simulink model "PV_SYSTEM_WITH_VARIOUS_MPPT"  (R2017a)
(part 4 of 6)

Inventec Energy IECS-6P68-190 | Inventec Energy IECS-6P69-190 | Inventec Energy IECS-6M68-195 | Inventec Energy IECS-6P68-195 | Inventec Energy IECS-6P69-195 | Inventec Energy IECS-6M69-200 | Inventec Energy IECS-6P68-200 | Inventec Energy IECS-6P69-200 | Inventec Energy IECS-6M69-205 | Inventec Energy IECS-6P68-205 | Inventec Energy IECS-6P69-205 | Inventec Energy IECS-6M69-210 | Inventec Energy IECS-6P69-210 | Inventec Energy IECS-6P6A-210 | Inventec Energy IECS-6M6A-215 | Inventec Energy IECS-6P69-215 | Inventec Energy IECS-6P6A-215 | Inventec Energy IECS-6M6A-220 | Inventec Energy IECS-6P69-220 | Inventec Energy IECS-6P6A-220 | Inventec Energy IECS-6M6A-225 | Inventec Energy IECS-6P69-225 | Inventec Energy IECS-6P6A-225 | Inventec Energy IECS-6M6A-230 | Inventec Energy IECS-6P69-230 | Inventec Energy IECS-6P6A-230 | Inventec Energy IECS-6M6A-235 | Inventec Energy IECS-6P6A-235 | Inventec Energy IECS-6M6A-240 | Inventec Energy IECS-6P6A-240 | Inventec Energy IECS-6M6A-245 | Inventec Energy IECS-6P6A-245 | Inventec Energy IECS-6M6A-250 | Inventec Energy IECS-6P6A-250 | Inventec Energy IECS-6M6A-255 | Inventec Energy IECS-6P6A-255 | Inventec Energy IECS-6M6A-260 | Inventec Energy IECS-6M6A-265 | Inventec Energy IECS-6M6A-270 | Inventec Energy IECS-6M6A-275 | Inventec Energy IECS-6P6C-275 | Inventec Energy IECS-6P6C-280 | Inventec Energy IECS-6M6C-285 | Inventec Energy IECS-6P6C-285 | Inventec Energy IECS-6M6C-290 | Inventec Energy IECS-6P6C-290 | Inventec Energy IECS-6M6C-295 | Inventec Energy IECS-6P6C-295 | Inventec Energy IECS-6M6C-300 | Inventec Energy IECS-6P6C-300 | Inventec Energy IECS-6M6C-305 | Inventec Energy IECS-6M6C-310 | Inventec Energy IECS-6M6C-315 | Inventec Energy IECS-6M6C-320 | Inventec Energy IECS-6M6C-325 | Inventec Energy IECS-6M6C-330 | Isofoton IS-210-32 | Isofoton IS-215-32 | Isofoton IS-220-32 | Isofoton ISF-235 | Isofoton ISF-240 | Isofoton ISF-245 | Isofoton ISF-245 Black | Isofoton ISF-245 Clear | Isofoton ISFT-245 | Isofoton ISF-250 | Isofoton ISF-250 Black | Isofoton ISF-250 Clear | Isofoton ISFT-250 | Isofoton ISF-255 | Isofoton ISF-255 Black | Isofoton ISF-255 Clear | Isofoton ISFT-255 | iTek iT-220 | iTek iT-225 | iTek iT-230 | iTek iT-235 | iTek iT-240 | Jetion Solar (China) JT175SAb | Jetion Solar (China) JT175SAb(Black) | Jetion Solar (China) JT180SAb | Jetion Solar (China) JT180SAb(Black) | Jetion Solar (China) JT185SAb | Jetion Solar (China) JT185SAb(Black) | Jetion Solar (China) JT190SAb | Jetion Solar (China) JT195SAb | Jetion Solar (China) JT220PCe | Jetion Solar (China) JT220PCe(Black) | Jetion Solar (China) JT225PCe | Jetion Solar (China) JT225PCe(Black) | Jetion Solar (China) JT230PCe | Jetion Solar (China) JT230PCe(Black) | Jetion Solar (China) JT230SCc | Jetion Solar (China) JT230SCc(Black) | Jetion Solar (China) JT235PCe | Jetion Solar (China) JT235PCe(Black) | Jetion Solar (China) JT235SCc | Jetion Solar (China) JT235SCc(Black) | Jetion Solar (China) JT240PCe | Jetion Solar (China) JT240PCe(Black) | Jetion Solar (China) JT240SCc | Jetion Solar (China) JT240SCc(Black) | Jetion Solar (China) JT245SCc | Jetion Solar (China) JT245SCc(Black) | Jetion Solar (China) JT250SCc | Jetion Solar (China) JT270PAe | Jetion Solar (China) JT270PAe(Black) | Jetion Solar (China) JT270SAc | Jetion Solar (China) JT270SAc(Black) | Jetion Solar (China) JT275PAe | Jetion Solar (China) JT275PAe(Black) | Jetion Solar (China) JT275SAc | Jetion Solar (China) JT275SAc(Black) | Jetion Solar (China) JT280PAe | Jetion Solar (China) JT280PAe(Black) | Jetion Solar (China) JT280SAc | Jetion Solar (China) JT280SAc(Black) | Jetion Solar (China) JT285PAe | Jetion Solar (China) JT285PAe(Black) | Jetion Solar (China) JT285SAc | Jetion Solar (China) JT285SAc(Black) | Jetion Solar (China) JT290PAe | Jetion Solar (China) JT290PAe(Black) | Jetion Solar (China) JT290SAc | Jetion Solar (China) JT290SAc(Black) | Jiangsu Aide Solar Energy Technology AD160M5-Aa | Jiangsu Aide Solar Energy Technology AD165M5-Aa | Jiangsu Aide Solar Energy Technology AD170M5-Aa | Jiangsu Aide Solar Energy Technology AD175M5-Aa | Jiangsu Aide Solar Energy Technology AD180M5-Aa | Jiangsu Aide Solar Energy Technology AD185M5-Aa | Jiangsu Aide Solar Energy Technology AD190M5-Aa | Jiangsu Aide Solar Energy Technology AD190P6-Ac | Jiangsu Aide Solar Energy Technology AD195M5-Aa | Jiangsu Aide Solar Energy Technology AD195P6-Ac | Jiangsu Aide Solar Energy Technology AD200M5-Aa | Jiangsu Aide Solar Energy Technology AD200P6-Ac | Jiangsu Aide Solar Energy Technology AD205P6-Ac | Jiangsu Aide Solar Energy Technology AD210P6-Ac | Jiangsu Aide Solar Energy Technology AD210P6-Bc | Jiangsu Aide Solar Energy Technology AD215P6-Ab | Jiangsu Aide Solar Energy Technology AD220P6-Ab | Jiangsu Aide Solar Energy Technology AD220P6-Bb | Jiangsu Aide Solar Energy Technology AD225P6-Ab | Jiangsu Aide Solar Energy Technology AD230M6-Ab | Jiangsu Aide Solar Energy Technology AD230P6-Ab | Jiangsu Aide Solar Energy Technology AD230P6-Bb | Jiangsu Aide Solar Energy Technology AD235M6-Ab | Jiangsu Aide Solar Energy Technology AD235P6-Ab | Jiangsu Aide Solar Energy Technology AD235P6-Bb | Jiangsu Aide Solar Energy Technology AD240M6-Ab | Jiangsu Aide Solar Energy Technology AD240P6-Ab | Jiangsu Aide Solar Energy Technology AD240P6-Bb | Jiangsu Aide Solar Energy Technology AD245M6-Ab | Jiangsu Aide Solar Energy Technology AD245P6-Ab | Jiangsu Aide Solar Energy Technology AD250M6-Ab | Jiangsu Aide Solar Energy Technology AD250P6-Ab | Jiangsu Aide Solar Energy Technology AD255M6-Ab | Jiangsu Aide Solar Energy Technology AD255P6-Ab | Jiangsu Aide Solar Energy Technology AD260M6-Ab | Jiangsu Aide Solar Energy Technology AD260P6-Ab | Jiangsu Aide Solar Energy Technology AD265M6-Ab | Jiangsu Aide Solar Energy Technology AD275M6-Aa | Jiangsu Aide Solar Energy Technology AD275P6-Aa | Jiangsu Aide Solar Energy Technology AD280M6-Aa | Jiangsu Aide Solar Energy Technology AD280P6-Aa | Jiangsu Aide Solar Energy Technology AD285M6-Aa | Jiangsu Aide Solar Energy Technology AD285P6-Aa | Jiangsu Aide Solar Energy Technology AD290M6-Aa | Jiangsu Aide Solar Energy Technology AD290P6-Aa | Jiangsu Aide Solar Energy Technology AD295M6-Aa | Jiangsu Aide Solar Energy Technology AD295P6-Aa | Jiangsu Aide Solar Energy Technology AD300M6-Aa | Jiangsu Aide Solar Energy Technology AD300P6-Aa | Jiangsu Aide Solar Energy Technology AD305M6-Aa | Jiangsu Aide Solar Energy Technology AD305P6-Aa | Jiangsu Aide Solar Energy Technology AD310M6-Aa | Jiangsu Aide Solar Energy Technology AD310P6-Aa | Jiangsu Aide Solar Energy Technology AD315M6-Aa | Jiangsu Best Solar High-Tech BEST-170D-24 | Jiangsu Best Solar High-Tech BEST-175D-24 | Jiangsu Best Solar High-Tech BEST-180D-24 | Jiangsu Best Solar High-Tech BEST-190P-18 | Jiangsu Best Solar High-Tech BEST-200P-18 | Jiangsu Best Solar High-Tech BEST-210P-18 | Jiangsu Best Solar High-Tech BEST-210P-20 | Jiangsu Best Solar High-Tech BEST-220D-20 | Jiangsu Best Solar High-Tech BEST-220P-20 | Jiangsu Best Solar High-Tech BEST-230D-20 | Jiangsu Best Solar High-Tech BEST-230P-20 | Jiangsu Best Solar High-Tech BEST-240D-20 | Jiangsu Best Solar High-Tech BEST-260P-24 | Jiangsu Best Solar High-Tech BEST-270P-24 | Jiangsu Best Solar High-Tech BEST-280P-24 | Jiangsu Green Power PV GPM175-A-72 | Jiangsu Green Power PV GPM175-B-48 | Jiangsu Green Power PV GPM175P-B-48 | Jiangsu Green Power PV GPM180-A-72 | Jiangsu Green Power PV GPM180-B-48 | Jiangsu Green Power PV GPM180P-B-48 | Jiangsu Green Power PV GPM185-A-72 | Jiangsu Green Power PV GPM185-B-48 | Jiangsu Green Power PV GPM185P-B-48 | Jiangsu Green Power PV GPM190-B-54 | Jiangsu Green Power PV GPM190P-B-54 | Jiangsu Green Power PV GPM195-B-54 | Jiangsu Green Power PV GPM195P-B-54 | Jiangsu Green Power PV GPM200-B-54 | Jiangsu Green Power PV GPM200P-B-54 | Jiangsu Green Power PV GPM205-B-54 | Jiangsu Green Power PV GPM205P-B-54 | Jiangsu Green Power PV GPM210-B-54 | Jiangsu Green Power PV GPM210P-B-54 | Jiangsu Green Power PV GPM210P-B-60 | Jiangsu Green Power PV GPM215P-B-60 | Jiangsu Green Power PV GPM220-B-60 | Jiangsu Green Power PV GPM220P-B-60 | Jiangsu Green Power PV GPM225-B-60 | Jiangsu Green Power PV GPM225P-B-60 | Jiangsu Green Power PV GPM230-B-60 | Jiangsu Green Power PV GPM230P-B-60 | Jiangsu Green Power PV GPM235-B-60 | Jiangsu Green Power PV GPM240-B-60 | Jiangsu JiaSheng Photovoltaic Technology JS140M36-12V | Jiangsu JiaSheng Photovoltaic Technology JS140P36-12V | Jiangsu JiaSheng Photovoltaic Technology JS145M36-12V | Jiangsu JiaSheng Photovoltaic Technology JS145P36-12V | Jiangsu JiaSheng Photovoltaic Technology JS180D72-24V | Jiangsu JiaSheng Photovoltaic Technology JS185D72-24V | Jiangsu JiaSheng Photovoltaic Technology JS190D72-24V | Jiangsu JiaSheng Photovoltaic Technology JS195D72-24V | Jiangsu JiaSheng Photovoltaic Technology JS220P60-24V | Jiangsu JiaSheng Photovoltaic Technology JS225P60-24V | Jiangsu JiaSheng Photovoltaic Technology JS230M60-24V | Jiangsu JiaSheng Photovoltaic Technology JS230P60-24V | Jiangsu JiaSheng Photovoltaic Technology JS235M60-24V | Jiangsu JiaSheng Photovoltaic Technology JS235P60-24V | Jiangsu JiaSheng Photovoltaic Technology JS240M60-24V | Jiangsu JiaSheng Photovoltaic Technology JS240P60-24V | Jiangsu JiaSheng Photovoltaic Technology JS245M60-24V | Jiangsu JiaSheng Photovoltaic Technology JS250M60-24V | Jiangsu JiaSheng Photovoltaic Technology JS255M60-24V | Jiangsu JiaSheng Photovoltaic Technology JS255P72-24V | Jiangsu JiaSheng Photovoltaic Technology JS260M60-24V | Jiangsu JiaSheng Photovoltaic Technology JS260M72-24V | Jiangsu JiaSheng Photovoltaic Technology JS260P72-24V | Jiangsu JiaSheng Photovoltaic Technology JS265M72-24V | Jiangsu JiaSheng Photovoltaic Technology JS265P72-24V | Jiangsu JiaSheng Photovoltaic Technology JS270M72-24V | Jiangsu JiaSheng Photovoltaic Technology JS270P72-24V | Jiangsu JiaSheng Photovoltaic Technology JS275M72-24V | Jiangsu JiaSheng Photovoltaic Technology JS275P72-24V | Jiangsu JiaSheng Photovoltaic Technology JS280M72-24V | Jiangsu JiaSheng Photovoltaic Technology JS280P72-24V | Jiangsu JiaSheng Photovoltaic Technology JS290M72-24V | Jiangsu JiaSheng Photovoltaic Technology JS290P72-24V | Jiangsu JiaSheng Photovoltaic Technology JS300M72-24V | Jiangsu JiaSheng Photovoltaic Technology JS300P72-24V | Jiangsu Prefersolar Photovoltaic PS-175M | Jiangsu Prefersolar Photovoltaic PS-180M | Jiangsu Prefersolar Photovoltaic PS-185M | Jiangsu Prefersolar Photovoltaic PS-230M | Jiangsu Prefersolar Photovoltaic PS-235M | Jiangsu Prefersolar Photovoltaic PS-240M | Jiangsu Prefersolar Photovoltaic PS-245M | Jiangsu Prefersolar Photovoltaic PS-250M | Jiangsu Runda PV RS185M-72 | Jiangsu Runda PV RS190M-72 | Jiangsu Runda PV RS215P-60 | Jiangsu Runda PV RS220P-60 | Jiangsu Runda PV RS225P-60 | Jiangsu Runda PV RS230M-96 | Jiangsu Runda PV RS230P-60 | Jiangsu Runda PV RS235M-96 | Jiangsu Runda PV RS235P-60 | Jiangsu Runda PV RS240M-96 | Jiangsu Runda PV RS245M-96 | Jiangsu Runda PV RS250M-96 | Jiangsu Sainty Machinery GES-M165 | Jiangsu Sainty Machinery GES-5M170 | Jiangsu Sainty Machinery GES-M170 | Jiangsu Sainty Machinery GES-5M175 | Jiangsu Sainty Machinery GES-M175 | Jiangsu Sainty Machinery GES-5M180 | Jiangsu Sainty Machinery GES-M180 | Jiangsu Sainty Machinery GES-5M185 | Jiangsu Sainty Machinery GES-5M190 | Jiangsu Sainty Machinery GES-6M190 | Jiangsu Sainty Machinery GES-5M195 | Jiangsu Sainty Machinery GES-6M195 | Jiangsu Sainty Machinery GES-6M200 | Jiangsu Sainty Machinery GES-P200 | Jiangsu Sainty Machinery GES-6M205 | Jiangsu Sainty Machinery GES-6M210 | Jiangsu Sainty Machinery GES-P210 | Jiangsu Sainty Machinery GES-6M220 | Jiangsu Sainty Machinery GES-P220 | Jiangsu Sainty Machinery GES-6M225 | Jiangsu Sainty Machinery GES-6P225 | Jiangsu Sainty Machinery GES-5M230 | Jiangsu Sainty Machinery GES-6M230 | Jiangsu Sainty Machinery GES-6P230 | Jiangsu Sainty Machinery GES-P230 | Jiangsu Sainty Machinery GES-5M235 | Jiangsu Sainty Machinery GES-6M235 | Jiangsu Sainty Machinery GES-6P235 | Jiangsu Sainty Machinery GES-5M240 | Jiangsu Sainty Machinery GES-6M240 | Jiangsu Sainty Machinery GES-6P240 | Jiangsu Sainty Machinery GES-P240 | Jiangsu Sainty Machinery GES-5M245 | Jiangsu Sainty Machinery GES-6M245 | Jiangsu Sainty Machinery GES-6P245 | Jiangsu Sainty Machinery GES-5M250 | Jiangsu Sainty Machinery GES-6M250 | Jiangsu Sainty Machinery GES-P250 | Jiangsu Sainty Machinery GES-5M255 | Jiangsu Sainty Machinery GES-6M255 | Jiangsu Sainty Machinery GES-6P255 | Jiangsu Sainty Machinery GES-6M260 | Jiangsu Sainty Machinery GES-6P260 | Jiangsu Sainty Machinery GES-P260 | Jiangsu Sainty Machinery GES-6M265 | Jiangsu Sainty Machinery GES-6P265 | Jiangsu Sainty Machinery GES-6M270 | Jiangsu Sainty Machinery GES-6P270 | Jiangsu Sainty Machinery GES-P270 | Jiangsu Sainty Machinery GES-6M275 | Jiangsu Sainty Machinery GES-6P275 | Jiangsu Sainty Machinery GES-6M280 | Jiangsu Sainty Machinery GES-6P280 | Jiangsu Sainty Machinery GES-P280 | Jiangsu Sainty Machinery GES-6M285 | Jiangsu Sainty Machinery GES-6P285 | Jiangsu Sainty Machinery GES-6M290 | Jiangsu Sainty Machinery GES-6P290 | Jiangsu Sainty Machinery GES-6M295 | Jiangsu Sainty Machinery GES-6P295 | Jiangsu Sainty Machinery GES-6M300 | Jiangsu Sainty Machinery GES-6P300 | Jiangsu Sainty Machinery GES-6M305 | Jiangsu Sainty Machinery GES-6M310 | Jiangsu Sainty Machinery GES-6M315 | Jiangsu Shunda PV-Tech SDM-170-(165)-72M | Jiangsu Shunda PV-Tech SDM-170-(170)-72M | Jiangsu Shunda PV-Tech SDM-170-(175)-72M | Jiangsu Shunda PV-Tech SDM-170-(180)-72M | Jiangsu Shunda PV-Tech SDM-170-(185)-72M | Jiangsu SunLink PV Technology SL180-24M170 | Jiangsu SunLink PV Technology SL180-24M175 | Jiangsu SunLink PV Technology SL180-24M180 | Jiangsu SunLink PV Technology SL180-24M185 | Jiangsu SunLink PV Technology SL180-24M190 | Jiangsu SunLink PV Technology SL180-24M195 | Jiangsu SunLink PV Technology SL220-20M200 | Jiangsu SunLink PV Technology SL220-20P200 | Jiangsu SunLink PV Technology SL220-20M205 | Jiangsu SunLink PV Technology SL220-20P205 | Jiangsu SunLink PV Technology SL220-20M210 | Jiangsu SunLink PV Technology SL220-20P210 | Jiangsu SunLink PV Technology SL220-20M215 | Jiangsu SunLink PV Technology SL220-20P215 | Jiangsu SunLink PV Technology SL220-20M220 | Jiangsu SunLink PV Technology SL220-20P220 | Jiangsu SunLink PV Technology SL240-32M220 | Jiangsu SunLink PV Technology SL220-20M225 | Jiangsu SunLink PV Technology SL220-20P225 | Jiangsu SunLink PV Technology SL240-32M225 | Jiangsu SunLink PV Technology SL220-20M230 | Jiangsu SunLink PV Technology SL220-20P230 | Jiangsu SunLink PV Technology SL240-32M230 | Jiangsu SunLink PV Technology SL220-20M235 | Jiangsu SunLink PV Technology SL220-20P235 | Jiangsu SunLink PV Technology SL240-32M235 | Jiangsu SunLink PV Technology SL220-20M240 | Jiangsu SunLink PV Technology SL220-20P240 | Jiangsu SunLink PV Technology SL240-32M240 | Jiangsu SunLink PV Technology SL220-20M245 | Jiangsu SunLink PV Technology SL240-32M245 | Jiangsu SunLink PV Technology SL220-20M250 | Jiangsu SunLink PV Technology SL240-32M250 | Jiangsu SunLink PV Technology SL220-20M255 | Jiangsu SunLink PV Technology SL240-32M255 | Jiangsu SunLink PV Technology SL220-20M260 | Jiangsu SunLink PV Technology SL280-24M260 | Jiangsu SunLink PV Technology SL280-24P260 | Jiangsu SunLink PV Technology SL280-24M265 | Jiangsu SunLink PV Technology SL280-24P265 | Jiangsu SunLink PV Technology SL280-24M270 | Jiangsu SunLink PV Technology SL280-24P270 | Jiangsu SunLink PV Technology SL280-24M275 | Jiangsu SunLink PV Technology SL280-24P275 | Jiangsu SunLink PV Technology SL280-24M280 | Jiangsu SunLink PV Technology SL280-24P280 | Jiangsu SunLink PV Technology SL280-24M285 | Jiangsu SunLink PV Technology SL280-24P285 | Jiangsu SunLink PV Technology SL280-24M290 | Jiangsu SunLink PV Technology SL280-24P290 | Jiangsu SunLink PV Technology SL280-24M295 | Jiangsu SunLink PV Technology SL280-24P295 | Jiangsu Wanfeng PV WF175M-01E | Jiangsu Wanfeng PV WF180M-01E | Jiangsu Wanfeng PV WF185M-01E | Jiangsu Wanfeng PV WF200P-02B | Jiangsu Wanfeng PV WF205P-02B | Jiangsu Wanfeng PV WF210P-02B | Jiangsu Wanfeng PV WF215P-02B | Jiangsu Wanfeng PV WF220P-02B | Jiangsu Wanfeng PV WF225P-02B | Jiangsu Wanfeng PV WF230P-02B | Jiangsu Wanfeng PV WF240P-02A | Jiangsu Wanfeng PV WF245P-02A | Jiangsu Wanfeng PV WF250P-02A | Jiangsu Wanfeng PV WF255P-02A | Jiangsu Wanfeng PV WF260P-02A | Jiangsu Wanfeng PV WF265P-02A | Jiangsu Wanfeng PV WF270P-02A | Jiangsu Wanfeng PV WF275P-02A | Jiangsu Wanfeng PV WF280P-02A | Jiangxi Best Solar High-Tech BEST-170D-24 | Jiangxi Best Solar High-Tech BEST-175D-24 | Jiangxi Best Solar High-Tech BEST-180D-24 | Jiangxi Best Solar High-Tech BEST-190P-18 | Jiangxi Best Solar High-Tech BEST-200P-18 | Jiangxi Best Solar High-Tech BEST-210P-18 | Jiangxi Best Solar High-Tech BEST-210P-20 | Jiangxi Best Solar High-Tech BEST-220D-20 | Jiangxi Best Solar High-Tech BEST-220P-20 | Jiangxi Best Solar High-Tech BEST-230D-20 | Jiangxi Best Solar High-Tech BEST-230P-20 | Jiangxi Best Solar High-Tech BEST-240D-20 | Jiangxi Best Solar High-Tech BEST-260P-24 | Jiangxi Best Solar High-Tech BEST-270P-24 | Jiangxi Best Solar High-Tech BEST-280P-24 | Jiangyin Hareon Power HR-115W-17V | Jiangyin Hareon Power HR-120W-17V | Jiangyin Hareon Power HR-125W-17V | Jiangyin Hareon Power HR-160W-24V | Jiangyin Hareon Power HR-165W-24V | Jiangyin Hareon Power HR-170W-24V | Jiangyin Hareon Power HR-175W-24V | Jiangyin Hareon Power HR-180W-24V | Jiangyin Hareon Power HR-185W-24V | Jiangyin Hareon Power HR-190W-24V | Jiangyin Hareon Power HR-195W-24V | Jiangyin Hareon Power HR-200W-18V | Jiangyin Hareon Power HR-200W-24V | Jiangyin Hareon Power HR-205W-18V | Jiangyin Hareon Power HR-210W-18V | Jiangyin Hareon Power HR-215W-18V | Jiangyin Hareon Power HR220D6P-3 | Jiangyin Hareon Power HR-220W-18V | Jiangyin Hareon Power HR225D6P-3 | Jiangyin Hareon Power HR-225P-18-Bb | Jiangyin Hareon Power HR-225P-18-Bbp | Jiangyin Hareon Power HR-225W-18V | Jiangyin Hareon Power HR230D6P-3 | Jiangyin Hareon Power HR-230P-18-Bb | Jiangyin Hareon Power HR-230P-18-Bbp | Jiangyin Hareon Power HR-230W-18V | Jiangyin Hareon Power HR235D6P-3 | Jiangyin Hareon Power HR-235P-18-Bb | Jiangyin Hareon Power HR-235P-18-Bbp | Jiangyin Hareon Power HR-235W-18V | Jiangyin Hareon Power HR-240P-18-Bb | Jiangyin Hareon Power HR-240P-18-Bbp | Jiangyin Hareon Power HR-240W-18V | Jiangyin Hareon Power HR-245P-18-Bb | Jiangyin Hareon Power HR-245P-18-Bbp | Jiangyin Hareon Power HR-250-18-Cb | Jiangyin Hareon Power HR-250P-18-Bb | Jiangyin Hareon Power HR-250P-18-Bbp | Jiangyin Hareon Power HR-255-18-Cb | Jiangyin Hareon Power HR-255P-18-Bb | Jiangyin Hareon Power HR-255P-18-Bbp | Jiangyin Hareon Power HR-260-18-Cb | Jiangyin Hareon Power HR-260P-18-Bb | Jiangyin Hareon Power HR-260P-18-Bbp | Jiangyin Hareon Power HR-265-18-Cb | Jiangyin Hareon Power HR-265P-18-Bb | Jiangyin Hareon Power HR-265P-18-Bbp | Jiangyin Hareon Power HR-270-18-Cb | Jiangyin Hareon Power HR-270P-24-Ba | Jiangyin Hareon Power HR-270P-24-Bap | Jiangyin Hareon Power HR-275P-24-Ba | Jiangyin Hareon Power HR-275P-24-Bap | Jiangyin Hareon Power HR-280P-24-Ba | Jiangyin Hareon Power HR-280P-24-Bap | Jiangyin Hareon Power HR-285P-24-Ba | Jiangyin Hareon Power HR-285P-24-Bap | Jiangyin Hareon Power HR-290P-24-Ba | Jiangyin Hareon Power HR-290P-24-Bap | Jiangyin Hareon Power HR-295-24-Ca | Jiangyin Hareon Power HR-295P-24-Ba | Jiangyin Hareon Power HR-295P-24-Bap | Jiangyin Hareon Power HR-300-24-Ca | Jiangyin Hareon Power HR-300P-24-Ba | Jiangyin Hareon Power HR-300P-24-Bap | Jiangyin Hareon Power HR-305-24-Ca | Jiangyin Hareon Power HR-305P-24-Ba | Jiangyin Hareon Power HR-305P-24-Bap | Jiangyin Hareon Power HR-310-24-Ca | Jiangyin Hareon Power HR-310P-24-Ba | Jiangyin Hareon Power HR-310P-24-Bap | Jiangyin Hareon Power HR-315-24-Ca | Jiangyin Hareon Power HR-315P-24-Ba | Jiangyin Hareon Power HR-315P-24-Bap | Jiangyin Hareon Power HR-320P-24-Ba | Jiangyin Hareon Power HR-320P-24-Bap | Jiangyin Jetion Science and Technology JT210PCe | Jiangyin Jetion Science and Technology JT215PCe | Jiawei Solarchina (Shenzhen) JW-G2300-MD6660P-1 | Jiawei Solarchina (Shenzhen) JW-G2300-QC6660P-1 | Jingao Solar JAM5(L)-175 | Jingao Solar JAM5(L)-180 | Jingao Solar JAM5(L)-185 | Jingao Solar JAM6-200 | Jingao Solar JAP6-200 | Jingao Solar JAM6-205 | Jingao Solar JAP6-205 | Jingao Solar JAM6-210 | Jingao Solar JAP6-210 | Jingao Solar JAM6-215 | Jingao Solar JAP6-215 | Jingao Solar JAM6-220 | Jingao Solar JAP6-220 | Jingao Solar JAM6-225 | Jingao Solar JAP6-225 | Jingao Solar JAM6-230 | Jingao Solar JAP6-230 | Jingao Solar JAM6-235 | Jingao Solar JAP6-235 | Jingao Solar JAM6-240 | Jingao Solar JAP6-240 | Jinko Solar JKM170M-72B | Jinko Solar JKM175M-72 | Jinko Solar JKM175M-72B | Jinko Solar JKM180M-72 | Jinko Solar JKM180M-72B | Jinko Solar JKM185M-72 | Jinko Solar JKM185M-72B | Jinko Solar JKM190M-72 | Jinko Solar JKM190M-72B | Jinko Solar JKM195M-72 | Jinko Solar JKM195M-72B | Jinko Solar JKM200M-60B | Jinko Solar JKM200M-72 | Jinko Solar JKM200M-72B | Jinko Solar JKM200P-60B | Jinko Solar JKM205M-60B | Jinko Solar JKM205M-72 | Jinko Solar JKM205M-72B | Jinko Solar JKM205P-60B | Jinko Solar JKM210M-60B | Jinko Solar JKM210P-60B | Jinko Solar JKM215M-60B | Jinko Solar JKM215P-60B | Jinko Solar JKM220M-60 | Jinko Solar JKM220M-60B | Jinko Solar JKM220P-60 | Jinko Solar JKM220P-60B | Jinko Solar JKM225M-60 | Jinko Solar JKM225M-60B | Jinko Solar JKM225P-60 | Jinko Solar JKM225P-60B | Jinko Solar JKM230M-60 | Jinko Solar JKM230M-60B | Jinko Solar JKM230P-60 | Jinko Solar JKM230P-60B | Jinko Solar JKM235M-60 | Jinko Solar JKM235M-60B | Jinko Solar JKM235P-60 | Jinko Solar JKM235P-60B | Jinko Solar JKM240M-60 | Jinko Solar JKM240M-60B | Jinko Solar JKM240P-60 | Jinko Solar JKM240P-60B | Jinko Solar JKM245M-60 | Jinko Solar JKM245M-60B | Jinko Solar JKM245P-60 | Jinko Solar JKM245P-60B | Jinko Solar JKM250M-60 | Jinko Solar JKM250M-72B | Jinko Solar JKM250P-60 | Jinko Solar JKM250P-72 | Jinko Solar JKM250P-72B | Jinko Solar JKM255M-60 | Jinko Solar JKM255M-72B | Jinko Solar JKM255M-96 | Jinko Solar JKM255P-60 | Jinko Solar JKM255P-72 | Jinko Solar JKM255P-72B | Jinko Solar JKM260M-72B | Jinko Solar JKM260M-96 | Jinko Solar JKM260P-72 | Jinko Solar JKM260P-72B | Jinko Solar JKM265M-72B | Jinko Solar JKM265M-96 | Jinko Solar JKM265P-72 | Jinko Solar JKM265P-72B | Jinko Solar JKM270M-72 | Jinko Solar JKM270M-72B | Jinko Solar JKM270M-96 | Jinko Solar JKM270P-72 | Jinko Solar JKM270P-72B | Jinko Solar JKM275M-72 | Jinko Solar JKM275M-72B | Jinko Solar JKM275M-96 | Jinko Solar JKM275P-72 | Jinko Solar JKM275P-72B | Jinko Solar JKM280M-72 | Jinko Solar JKM280M-72B | Jinko Solar JKM280M-96 | Jinko Solar JKM280P-72 | Jinko Solar JKM280P-72B | Jinko Solar JKM285M-72 | Jinko Solar JKM285M-72B | Jinko Solar JKM285P-72 | Jinko Solar JKM285P-72B | Jinko Solar JKM290M-72 | Jinko Solar JKM290M-72B | Jinko Solar JKM290P-72 | Jinko Solar JKM290P-72B | Jinko Solar JKM295M-72 | Jinko Solar JKM295M-72B | Jinko Solar JKM295P-72 | Jinko Solar JKM295P-72B | Jinko Solar JKM300M-72 | Jinko Solar JKM305M-72 | Jinko Solar JKM305P-72 | Jinko Solar JKM310M-72 | Jinzhou Jinmao Photovoltaic Technology JMPV-5M-36-85 | Jinzhou Jinmao Photovoltaic Technology JMPV-5M-36-90 | Jinzhou Jinmao Photovoltaic Technology JMPV-5M-36-95 | Jinzhou Jinmao Photovoltaic Technology JMPV-5M-72-165 | Jinzhou Jinmao Photovoltaic Technology JMPV-5M-72-170 | Jinzhou Jinmao Photovoltaic Technology JMPV-5M-72-175 | Jinzhou Jinmao Photovoltaic Technology JMPV-5M-72-180 | Jinzhou Jinmao Photovoltaic Technology JMPV-5M-72-185 | Jinzhou Jinmao Photovoltaic Technology JMPV-5M-72-190 | Juli New Energy JLS155M | Juli New Energy JLS160M | Juli New Energy JLS165M | Juli New Energy JLS170M | Juli New Energy JLS175M | Juli New Energy JLS180M | Juli New Energy JLS200M | Juli New Energy JLS205M | Juli New Energy JLS210M | Juli New Energy JLS215P | Juli New Energy JLS220P | Juli New Energy JLS225P | Juli New Energy JLS230P | Jumao Photonic (Xiamen) JMP-85W-S5-G | Jumao Photonic (Xiamen) JMP-160W-S5-G | Jumao Photonic (Xiamen) JMP-170W-S5-G | Jumao Photonic (Xiamen) JMP-210W-M6-G | Jumao Photonic (Xiamen) JMP-215W-M6-G | Jumao Photonic (Xiamen) JMP-220W-M6-G | Jumao Photonic (Xiamen) JMP-225W-M6-G | Jumao Photonic (Xiamen) JMP-230W-M6-G | Kaneka G-SA060 | Kaneka GSA221 | Kaneka U-SA105 | Kaneka U-SA110 | KD Solar KD-20012A2 | KD Solar KD-20013A2 | KD Solar KD-20512A2 | KD Solar KD-20513A2 | KD Solar KD-21012A2 | KD Solar KD-21013A2 | KD Solar KD-21512A2 | KD Solar KD-21513A2 | KD Solar KD-22012A2 | KD Solar KD-22013A2 | KD Solar KD-22512A2 | KD Solar KD-22513A2 | KD Solar KD-23012A2 | KD Solar KD-23013A2 | KD Solar KD-23512A2 | KD Solar KD-24012A2 | Kenmec Mechanical Engineering TKSE-13001 | Kenmec Mechanical Engineering TKSE-13501 | Kenmec Mechanical Engineering TKSE-14001 | Kenmec Mechanical Engineering TKSE-14501 | Kenmec Mechanical Engineering TKSD-15001 | Kenmec Mechanical Engineering TKSD-15501 | Kenmec Mechanical Engineering TKSD-16001 | Kenmec Mechanical Engineering TKSD-16501 | Kenmec Mechanical Engineering TKSC-17001 | Kenmec Mechanical Engineering TKSD-17001 | Kenmec Mechanical Engineering TKSC-17501 | Kenmec Mechanical Engineering TKSC-18001 | Kenmec Mechanical Engineering TKSC-18501 | Kenmec Mechanical Engineering TKSC-19001 | Kenmec Mechanical Engineering TKSC-19501 | Kenmec Mechanical Engineering TKSB-20001 | Kenmec Mechanical Engineering TKSB-20501 | Kenmec Mechanical Engineering TKSB-21001 | Kenmec Mechanical Engineering TKSB-21501 | Kenmec Mechanical Engineering TKSA-22001 | Kenmec Mechanical Engineering TKSB-22001 | Kenmec Mechanical Engineering TKSA-22501 | Kenmec Mechanical Engineering TKSA-23001 | Kenmec Mechanical Engineering TKSA-23501 | Kenmec Mechanical Engineering TKSA-24001 | Kenmec Mechanical Engineering TKSA-24501 | Kenmec Mechanical Engineering TKSA-25001 | Kenmec Mechanical Engineering TKSG-25001 | Kenmec Mechanical Engineering TKSA-25501 | Kenmec Mechanical Engineering TKSG-25501 | Kenmec Mechanical Engineering TKSA-26001 | Kenmec Mechanical Engineering TKSG-26001 | Kenmec Mechanical Engineering TKSG-26501 | Kenmec Mechanical Engineering TKSG-27001 | Kenmec Mechanical Engineering TKSG-27501 | Kenmec Mechanical Engineering TKSG-28001 | Kenmec Mechanical Engineering TKSG-28501 | Kenmec Mechanical Engineering TKSG-29001 | Kenmec Mechanical Engineering TKSG-29501 | Kenmec Mechanical Engineering TKSG-30001 | Kenmec Mechanical Engineering TKSG-30501 | Kenmec Mechanical Engineering TKSG-31001 | Kenmec Mechanical Engineering TKSG-31501 | Kenmos Photovoltaic aTT-50W-02 | Kinve Solar Power KV170-72M | Kinve Solar Power KV175-72M | Kinve Solar Power KV180-72M | KISCO S91E | KISCO S92E | KISCO S93E | KISCO S94E | KISCO S95E | KISCO S96E | KISCO S97E | KISCO S98E | KISCO S99E | KISCO S100E | KISCO S101E | KISCO GETWATT 224P-A1U | KISCO GETWATT 225P-A1U | KISCO GETWATT 226P-A1U | KISCO GETWATT 227P-A1U | KISCO GETWATT 228P-A1U | KISCO GETWATT 229P-A1U | KISCO GETWATT 230P-A1U | KISCO GETWATT 231P-A1U | KISCO GETWATT 232P-A1U | KISCO GETWATT 233P-A1U | KISCO GETWATT 234P-A1U | KISCO GETWATT 235P-A1U | KISCO GETWATT 236P-A1U | KISCO GETWATT 237P-A1U | KISCO GETWATT 238M-A1U | KISCO GETWATT 238P-A1U | KISCO GETWATT 239M-A1U | KISCO GETWATT 239P-A1U | KISCO GETWATT 240M-A1U | KISCO GETWATT 240M-C1U | KISCO GETWATT 240P-A1U | KISCO GETWATT 241M-A1U | KISCO GETWATT 241M-C1U | KISCO GETWATT 241P-A1U | KISCO GETWATT 242M-A1U | KISCO GETWATT 242M-C1U | KISCO GETWATT 242P-A1U | KISCO GETWATT 243M-A1U | KISCO GETWATT 243M-C1U | KISCO GETWATT 243P-A1U | KISCO GETWATT 244M-A1U | KISCO GETWATT 244M-C1U | KISCO GETWATT 244P-A1U | KISCO GETWATT 245M-A1U | KISCO GETWATT 245M-C1U | KISCO GETWATT 245P-A1U | KISCO GETWATT 246M-A1U | KISCO GETWATT 246M-C1U | KISCO GETWATT 247M-A1U | KISCO GETWATT 247M-C1U | KISCO GETWATT 248M-A1U | KISCO GETWATT 248M-C1U | KISCO GETWATT 249M-A1U | KISCO GETWATT 249M-C1U | KISCO GETWATT 250M-A1U | KISCO GETWATT 250M-C1U | KISCO GETWATT 251M-A1U | KISCO GETWATT 251M-C1U | KISCO GETWATT 252M-A1U | KISCO GETWATT 252M-C1U | KISCO GETWATT 253M-A1U | KISCO GETWATT 253M-C1U | KISCO GETWATT 254M-A1U | KISCO GETWATT 254M-C1U | KISCO GETWATT 255M-A1U | KISCO GETWATT 255M-C1U | KISCO GETWATT 256M-A1U | KISCO GETWATT 257M-A1U | KISCO GETWATT 258M-A1U | KISCO GETWATT 259M-A1U | KISCO GETWATT 260M-A1U | KISCO GETWATT 261M-A1U | KISCO GETWATT 262M-A1U | Konca Solar Cell KC5M-170a | Konca Solar Cell KC5M-175a | Konca Solar Cell KC5M-180a | Konca Solar Cell KC6P-215b | Konca Solar Cell KC6P-220b | Konca Solar Cell KC6P-225b | Konca Solar Cell KC6P-230b | Konca Solar Cell KC6P-235b | Kyocera Solar SU53BU | Kyocera Solar KC130GT | Kyocera Solar KC130TM | Kyocera Solar KD130GX-L | Kyocera Solar KD130GX-LFBS | Kyocera Solar KD130GX-LP | Kyocera Solar KD135GX-L | Kyocera Solar KD135GX-LFBS | Kyocera Solar KD135GX-LP | Kyocera Solar KD135GX-LPU | Kyocera Solar KD140GX-LFBS | Kyocera Solar KC175GT | Kyocera Solar KD180GX-L | Kyocera Solar KD180GX-LFBS | Kyocera Solar KD180GX-LP | Kyocera Solar KD185GX-LFBS | Kyocera Solar KD185GX-LPU | Kyocera Solar KD190GX-LFBS | Kyocera Solar KC200GT | Kyocera Solar KD200GX-LPU | Kyocera Solar KD205GX-L | Kyocera Solar KD205GX-LFBS | Kyocera Solar KD205GX-LP | Kyocera Solar KD205GX-LPU | Kyocera Solar KD210GX-L | Kyocera Solar KD210GX-LFBS | Kyocera Solar KD210GX-LP | Kyocera Solar KD210GX-LPU | Kyocera Solar KD215GX-LFBS | Kyocera Solar KD215GX-LPU | Kyocera Solar KD220GX-LFBS | Kyocera Solar KD225GX-LFB | Kyocera Solar KD225GX-LFBS | Kyocera Solar KD225GX-LPB | Kyocera Solar KD230GX-LFB | Kyocera Solar KD230GX-LPB | Kyocera Solar KD235GX-LFB | Kyocera Solar KD235GX-LPB | Kyocera Solar KD240GX-LFB | Kyocera Solar KD240GX-LFB2 | Kyocera Solar KD240GX-LPB | Kyocera Solar KD240GX-LPB2 | Kyocera Solar KD245GX-LFB | Kyocera Solar KD245GX-LFB2 | Kyocera Solar KD245GX-LPB | Kyocera Solar KD245GX-LPB2 | Kyocera Solar KD250GX-LFB | Kyocera Solar KD250GX-LFB2 | Kyocera Solar KD250GX-LPB | Kyocera Solar KD250GX-LPB2 | Kyocera Solar KD300GX-LFB | Kyocera Solar KD300GX-LPB | Kyocera Solar KD305GX-LFB | Kyocera Solar KD305GX-LPB | Kyocera Solar KD310GX-LFB | Kyocera Solar KD310GX-LPB | Kyocera Solar KD315GX-LFB | Kyocera Solar KD315GX-LPB | Kyocera Solar KD320GX-LFB | Kyocera Solar KD320GX-LPB | Kyocera Solar KD325GX-LFB | Kyocera Solar KD325GX-LPB | Kyung Won KWL-210 S | Kyung Won KWL-220 S | Kyung Won KWL-230 S | Kyung Won KWL-240 S | Kyung Won KWL-250 S | LG Electronics LG210P1C-G2 | LG Electronics LG210P1W-G1 | LG Electronics LG215P1C-G2 | LG Electronics LG215P1W | LG Electronics LG215P1W-G1 | LG Electronics LG220M1C-G2 | LG Electronics LG220P1C-G2 | LG Electronics LG220P1W | LG Electronics LG220P1W-G1 | LG Electronics LG220R1C-G2 | LG Electronics LG220R1W-G2 | LG Electronics LG225M1C-G2 | LG Electronics LG225P1C-G2 | LG Electronics LG225P1W | LG Electronics LG225P1W-G1 | LG Electronics LG225R1C-G2 | LG Electronics LG225R1W-G2 | LG Electronics LG230M1C-G2 | LG Electronics LG230P1C-G2 | LG Electronics LG230P1W | LG Electronics LG230P1W-G1 | LG Electronics LG230R1C-G2 | LG Electronics LG230R1W-G2 | LG Electronics LG235M1C-G2 | LG Electronics LG235P1W | LG Electronics LG235R1C-G2 | LG Electronics LG235R1W-G2 | LG Electronics LG240M1C-G2 | LG Electronics LG240R1C-G2 | LG Electronics LG240R1W-G2 | LG Electronics LG240S1C-G2 | LG Electronics LG240S1K-G3 | LG Electronics LG245M1C-G2 | LG Electronics LG245M1W-G2 | LG Electronics LG245S1C-G2 | LG Electronics LG245S1C-G3 | LG Electronics LG245S1K-G3 | LG Electronics LG250S1C-G2 | LG Electronics LG250S1C-G3 | LG Electronics LG250S1K-A3 | LG Electronics LG250S1K-G3 | LG Electronics LG255S1C-A3 | LG Electronics LG255S1C-G2 | LG Electronics LG255S1C-G3 | LG Electronics LG255S1K-A3 | LG Electronics LG255S1K-G3 | LG Electronics LG255S1W-A3 | LG Electronics LG260S1C-A3 | LG Electronics LG260S1C-G2 | LG Electronics LG260S1C-G3 | LG Electronics LG260S1K-A3 | LG Electronics LG260S1K-G3 | LG Electronics LG260S1W-A3 | LG Electronics LG260S1W-G2 | LG Electronics LG260S1W-G3 | LG Electronics LG265S1C-A3 | LG Electronics LG265S1C-G3 | LG Electronics LG265S1K-A3 | LG Electronics LG265S1W-A3 | LG Electronics LG265S1W-G3 | LG Electronics LG270N1C-G3 | LG Electronics LG270N1W-G3 | LG Electronics LG270S1C-A3 | LG Electronics LG270S1C-G3 | LG Electronics LG270S1W-A3 | LG Electronics LG270S1W-G3 | LG Electronics LG275N1C-G3 | LG Electronics LG275N1W-G3 | LG Electronics LG280N1C-G3 | LG Electronics LG280N1W-G3 | LG Electronics LG285N1C-G3 | LG Electronics LG285N1W-G3 | LG Electronics LG290N1C-G3 | LG Electronics LG290N1W-G3 | LG Electronics LG295N1C-G3 | LG Electronics LG295N1W-G3 | LG Electronics LG300N1C-G3 | LG Electronics LG300N1W-G3 | Lifeline Energy International LF-165WP | Lifeline Energy International LF-170WP | Lifeline Energy International LLE-5M170 | Lifeline Energy International LF-175WP | Lifeline Energy International LLE-5M175 | Lifeline Energy International LF-180WP | Lifeline Energy International LLE-5M180 | Lifeline Energy International LLE-5M185 | Lifeline Energy International LLE-5M190 | Lifeline Energy International LLE-5M195 | Lifeline Energy International LF-200WP | Lifeline Energy International LLE-6M205 | Lifeline Energy International LF-210WP | Lifeline Energy International LLE-6M210 | Lifeline Energy International LF-220WP | Lifeline Energy International LLE-6M220 | Lifeline Energy International LLE-6M225 | Lifeline Energy International LF-230WP | Lifeline Energy International LLE-6M230 | Lifeline Energy International LLE-6M235 | Lifeline Energy International LF-240WP | Lifeline Energy International LLE-6M240 | Lifeline Energy International LF-250WP | Lifeline Energy International LLE-6P255 | Lifeline Energy International LF-260WP | Lifeline Energy International LLE-6P260 | Lifeline Energy International LLE-6P265 | Lifeline Energy International LF-270WP | Lifeline Energy International LLE-6P270 | Lifeline Energy International LLE-6P275 | Lifeline Energy International LF-280WP | Lifeline Energy International LLE-6M280 | Lifeline Energy International LLE-6P280 | Lifeline Energy International LLE-6M285 | Lifeline Energy International LLE-6P285 | Lifeline Energy International LLE-6M290 | Lifeline Energy International LLE-6P290 | Lifeline Energy International LLE-6M295 | Lifeline Energy International LLE-6M300 | Lifeline Energy International LLE-6M305 | Lifeline Energy International LLE-6M310 | Lifeline Energy International LLE-6M315 | Lifeline Energy USA LFUS-200-p | Lifeline Energy USA LFUS-205-p | Lifeline Energy LF-215p-US | Lifeline Energy LF-220p-US | Lifeline Energy LF-225p-US | Lifeline Energy LF-230p-US | Lifeline Energy LF-235WP-US | Lifeline Energy LF-240WP-US | Lifeline Energy LF-245WP-US | Lifeline Energy LF-250WP-FLUS | Lifeline Energy LF-250WP-US | Lifeline Energy LFUS-250M | Lifeline Energy LF-260WP-FLUS | Lifeline Energy LFUS-300M | Lifeline Energy LF-335WP-US | Light Way Green New Energy LW165(23)P1310x990 | Light Way Green New Energy LW170(23)P1310x990 | Light Way Green New Energy LW175(23)P1310x990 | Light Way Green New Energy LW180(23)P1310x990 | Light Way Green New Energy LW185(23)P1310x990 | Light Way Green New Energy LW190(23)P1310x990 | Light Way Green New Energy LW200(29)P1650x990 | Light Way Green New Energy LW205(29)P1650x990 | Light Way Green New Energy LW210(29)P1650x990 | Light Way Green New Energy LW215(29)P1650x990 | Light Way Green New Energy LW220(29)P1650x990 | Light Way Green New Energy LW225(29)P1650x990 | Light Way Green New Energy LW230(29)P1650x990 | Light Way Green New Energy LW235(29)P1650x990 | Light Way Green New Energy LW240(29)P1650x990 | Light Way Green New Energy LW280(35)P1970990 | Light Way Green New Energy LW285(35)P1970990 | Light Way Green New Energy LW290(35)P1970990 | LS Industrial Systems PVM S228 | LS Industrial Systems PVM S229 | LS Industrial Systems PVM S230 | LS Industrial Systems PVM S231 | LS Industrial Systems PVM S232 | LS Industrial Systems PVM S233 | LS Industrial Systems PVM S234 | LS Industrial Systems PVM S235 | LS Industrial Systems PVM S236 | LS Industrial Systems PVM S237 | LS Industrial Systems PVM S238 | LS Industrial Systems PVM S239 | LS Industrial Systems PVM S240 | LS Industrial Systems PVM S241 | LS Industrial Systems PVM S242 | LS Industrial Systems PVM S243 | LS Industrial Systems PVM S244 | LS Industrial Systems PVM S245 | Lubi Electronics LE18P230 | Lubi Electronics LE18P240 | Lubi Electronics LE18P250 | Lucky Power Technology LPS-6P6A-220-B | Lucky Power Technology LPS-6P6A-225-B | Lucky Power Technology LPS-6P6A-230-B | Lucky Power Technology LPS-6P6A-235-B | Lucky Power Technology LPS-6P6A-240-B | LUMA Resources LRSS | Lumeta LEF028B | Lumeta LES028B | Lumeta LPP400A | Lumos LS175-72M-J | Lumos LSX175-72M-B | Lumos LSX175-72M-C | Lumos LSX175-72M-W | Lumos LS180-72M-J | Lumos LSX180-72M-B | Lumos LSX180-72M-C | Lumos LSX180-72M-W | Lumos LS185-72M | Lumos LS185-72M-J | Lumos LSX185-72M-B | Lumos LSX185-72M-C | Lumos LSX185-72M-W | Lumos LS190-72M | Lumos LS190-72M-J | Lumos LSX190-72M-B | Lumos LSX190-72M-C | Lumos LSX190-72M-W | Lumos LS195-72M-B | Lumos LS195-72M-J | Lumos LSX195-72M-B | Lumos LSX195-72M-C | Lumos LSX195-72M-W | Lumos LS200-72M-B | Lumos LS200-72M-J | Lumos LSX200-72M-B | Lumos LSX200-72M-C | Lumos LSX200-72M-W | Lumos LS205-72M-J | Lumos SST215-54M | Lumos SST215-54M-BB | Lumos LS220-60M | Lumos LS220-60M-J | Lumos LS220-60P-J | Lumos SST220-54M | Lumos SST220-54M-BB | Lumos SST220-60P | Lumos LS225-60M | Lumos LS225-60M-J | Lumos LS225-60P-J | Lumos LSX225-60M-B | Lumos LSX225-60M-C | Lumos LSX225-60M-W | Lumos SST225-54M | Lumos SST225-54M-BB | Lumos SST225-60P | Lumos LS230-60M | Lumos LS230-60M-J | Lumos LS230-60P-J | Lumos LSX230-60M-B | Lumos LSX230-60M-C | Lumos LSX230-60M-W | Lumos SST230-60P | Lumos LS235-60M | Lumos LS235-60M-J | Lumos LS235-60P-J | Lumos LS235PB | Lumos LS235PC | Lumos LSX235-60M-B | Lumos LSX235-60M-C | Lumos LSX235-60M-W | Lumos SST235-60M-BB | Lumos SST235-60P | Lumos LS240-60M | Lumos LS240-60M-B | Lumos LS240-60M-J | Lumos LS240-60P-B | Lumos LS240-60P-J | Lumos LS240PB | Lumos LS240PC | Lumos LSX240-60M-B | Lumos LSX240-60M-C | Lumos LSX240-60M-W | Lumos SST240-60M-BB | Lumos SST240-60P | Lumos LS245-60M | Lumos LS245-60M-A1 | Lumos LS245-60M-J | Lumos LS245-60P-J | Lumos LS245PB | Lumos LS245PC | Lumos LSX245-60M-B | Lumos LSX245-60M-C | Lumos LSX245-60M-W | Lumos SST245-60M-BB | Lumos LS250-60M | Lumos LS250-60M-A1 | Lumos LS250-60M-B | Lumos LS250-60M-J | Lumos LS250-72P-J | Lumos LSX250-60M-B | Lumos LSX250-60M-C | Lumos LSX250-60M-W | Lumos LS255-72P-J | Lumos LS260-72P-J | Lumos LS265-72M | Lumos LS265-72P-J | Lumos LS270-72M | Lumos LS270-72M-J | Lumos LS270-72P-J | Lumos LS275-72M | Lumos LS275-72M-J | Lumos LS275-72P | Lumos LS275-72P-J | Lumos LS280-72M | Lumos LS280-72M-J | Lumos LS280-72P | Lumos LS280-72P-B | Lumos LS280-72P-J | Lumos SST280-72M-BB | Lumos LS285-72M | Lumos LS285-72M-J | Lumos LS285-72P | Lumos LS285-72P-J | Lumos SST285-72M-BB | Lumos LS290-72M | Lumos LS290-72M-B | Lumos LS290-72M-J | Lumos LS290-72P | Lumos LS290-72P-J | Lumos SST290-72M-BB | Lumos LS295-72M | Lumos LS295-72M-A1 | Lumos LS295-72M-J | Lumos LS295-72P-J | Lumos SST295-72M-BB | Lumos LS300-72M | Lumos LS300-72M-A1 | Lumos LS300-72M-B | Lumos LS300-72M-J | Lumos LS305-72M-B | Lumos LS305-72M-J | Luxco LXP-2L270T | Luxco LXP-2L275T | Luxco LXP-2L280T | Luxco LXP-2L285T | Luxor Solar Solo Line 140M | Luxor Solar Solo Line 140P | Luxor Solar Solo Line 145M | Luxor Solar Solo Line 145P | Luxor Solar LX-180M-125-72+ | Luxor Solar LX-185M-125-72+ | Luxor Solar LX-190M-125-72+ | Luxor Solar LX-195M-125-72+ | Luxor Solar LX-220P-156-60+ | Luxor Solar LX-225P-156-60+ | Luxor Solar LX-230M-156-60+ | Luxor Solar LX-230P-156-60+ | Luxor Solar LX-235M-156-60+ | Luxor Solar LX-235P-156-60+ | Luxor Solar LX-240M-156-60+ | Luxor Solar LX-240P-156-60+ | Luxor Solar LX-245M-156-60+ | Luxor Solar LX-250M-156-60+ | Luxor Solar LX-255M-156-60+ | Luxor Solar LX-260M-156-60+ | Luxor Solar LX-260M-156-72+ | Luxor Solar LX-260P-156-72+ | Luxor Solar LX-265M-156-72+ | Luxor Solar LX-265P-156-72+ | Luxor Solar LX-270M-156-72+ | Luxor Solar LX-270P-156-72+ | Luxor Solar LX-275M-156-72+ | Luxor Solar LX-275P-156-72+ | Luxor Solar LX-280M-156-72+ | Luxor Solar LX-280P-156-72+ | Luxor Solar LX-290M-156-72+ | Luxor Solar LX-290P-156-72+ | Luxor Solar LX-300M-156-72+ | Luxor Solar LX-300P-156-72+ | Mage Solar USA Powertec Plus 190-5 MH-US | Mage Solar USA Powertec Plus 195-5MH-US | Mage Solar USA Powertec Plus 230-6 PH-US | Mage Solar USA Powertec Plus 230-6 PL | Mage Solar USA Powertec Plus 235-6 ML | Mage Solar USA Powertec Plus 235-6 PL | Mage Solar USA Powertec Plus 235-6PH-US | Mage Solar USA Powertec Plus 240-6 ML | Mage Solar USA Powertec Plus 240-6 PL | Mage Solar USA Powertec Plus 240-6 PNS | Mage Solar USA Powertec Plus 245-6 ML | Mage Solar USA Powertec Plus 245-6 MNBS | Mage Solar USA Powertec Plus 250-6 MNBS | Mage Solar USA Powertec Plus 250-6 MNCS | Mage Solar USA Powertec Plus 250-6 MNS | Mage Solar USA Powertec Plus 250-6 PL US | Mage Solar USA Powertec Plus 250-6 PL US AC | Mage Solar USA Powertec Plus 255-6 ML | Mage Solar USA Powertec Plus 290 - 6-72 PH | Mage Solar USA Powertec Plus 300-6 PL | MAGE Solar Powertec Plus 180-5 ME | MAGE Solar Powertec Plus 185-5 MH | MAGE Solar Powertec Plus 185-5MJB | MAGE Solar 190-5 MR | MAGE Solar Powertec Plus 190-5MH | MAGE Solar Powertec Plus 190-5MI | MAGE Solar Powertec Plus 195-5MH | MAGE Solar Powertec Plus 200-5MH | MAGE Solar Powertec Plus 220-6 PH | MAGE Solar Powertec Plus 220-6PI | MAGE Solar Powertec Plus 225-6PH | MAGE Solar Powertec Plus 230-6MI | MAGE Solar Powertec Plus 230-6MO | MAGE Solar Powertec Plus 230-6PE | MAGE Solar Powertec Plus 230-6PF | MAGE Solar Powertec Plus 230-6PH | MAGE Solar Powertec Plus 230-6PI | MAGE Solar Powertec Plus 230-6PJ | MAGE Solar Powertec Plus 230-6PO | MAGE Solar 235-6 PR | MAGE Solar Powertec Plus 235-6MF | MAGE Solar Powertec Plus 235-6MI | MAGE Solar Powertec Plus 235-6MO | MAGE Solar Powertec Plus 235-6PE | MAGE Solar Powertec Plus 235-6PH | MAGE Solar Powertec Plus 235-6PJ | MAGE Solar Powertec Plus 235-6PO | Mage Solar POWERTEC Plus 240 - 6 PL US | MAGE Solar Powertec Plus 240-6MF | MAGE Solar Powertec Plus 240-6MI | MAGE Solar Powertec Plus 240-6MO | MAGE Solar Powertec Plus 240-6PE | Mage Solar Powertec Plus 240-6PH | MAGE Solar Powertec Plus 240-6PJ | MAGE Solar Powertec Plus 240-6PO | MAGE Solar 245-5 MR | Mage Solar POWERTEC Plus 245 - 6 PL US AC | Mage Solar POWERTEC Plus 245 - 6PL US | MAGE Solar Powertec Plus 245-6 PL | MAGE Solar 250-5 MR | Mage Solar POWERTEC Plus 250 - 6 MN US | Mage Solar Powertec Plus 250-6 MH | MAGE Solar Powertec Plus 250-6 ML | MAGE Solar Powertec Plus 250-6 PL | MAGE Solar Powertec Plus 255-6 PL | MAGE Solar Powertec Plus 275-6 PL | MAGE Solar Powertec Plus 280-6 PL | MAGE Solar Powertec Plus 285-6 PL | MAGE Solar Powertec Plus 290-6 PL | Mage Solar Powertec Plus 290-6-72 PH | MAGE Solar Powertec Plus 295-6 PL | Mage Solar Powertec Plus 300-6-72 MH | Malaysian Solar Resources MYS-60P-B3-CF-235 | Malaysian Solar Resources MYS-60P-B3-CF-240 | Malaysian Solar Resources MYS-60P-B3-CF-245 | Martifer Solar MTS225P | MCV Technologies MCV-180 | MCV Technologies MCV-185 | MCV Technologies MCV-190 | MCV Technologies MCV-220 | MCV Technologies MCV-225 | MCV Technologies MCV-230 | MCV Technologies MCV-235 | MCV Technologies MCV-240 | MCV Technologies MCV-265 | MCV Technologies MCV-270 | MCV Technologies MCV-275 | MCV Technologies MCV-280 | MCV Technologies MCV-285 | MEMC Singapore MEMC-M230ACA-20 | MEMC Singapore MEMC-M230AMA-20 | MEMC Singapore MEMC-M230LCA-20 | MEMC Singapore MEMC-M230LMA-20 | MEMC Singapore MEMC-M235ACA-20 | MEMC Singapore MEMC-M235AMA-20 | MEMC Singapore MEMC-M240ACA-20 | MEMC Singapore MEMC-M240ACC-20 | MEMC Singapore MEMC-M240ACC-21 | MEMC Singapore MEMC-M240AIC-20 | MEMC Singapore MEMC-M240AIC-21 | MEMC Singapore MEMC-M240AMA-20 | MEMC Singapore MEMC-M240AMC-20 | MEMC Singapore MEMC-M240AMC-21 | MEMC Singapore MEMC-M240LCA-20 | MEMC Singapore MEMC-M240LCC-20 | MEMC Singapore MEMC-M240LCC-21 | MEMC Singapore MEMC-M240LIC-20 | MEMC Singapore MEMC-M240LIC-21 | MEMC Singapore MEMC-M240LMA-20 | MEMC Singapore MEMC-M240LMC-20 | MEMC Singapore MEMC-M240LMC-21 | MEMC Singapore MEMC-M245ACA-20 | MEMC Singapore MEMC-M245ACC-20 | MEMC Singapore MEMC-M245ACC-21 | MEMC Singapore MEMC-M245AIC-20 | MEMC Singapore MEMC-M245AIC-21 | MEMC Singapore MEMC-M245AMA-20 | MEMC Singapore MEMC-M245AMC-20 | MEMC Singapore MEMC-M245AMC-21 | MEMC Singapore MEMC-M245LCC-20 | MEMC Singapore MEMC-M245LCC-21 | MEMC Singapore MEMC-M245LIC-20 | MEMC Singapore MEMC-M245LIC-21 | MEMC Singapore MEMC-M245LMC-20 | MEMC Singapore MEMC-M245LMC-21 | MEMC Singapore SE-M245KZC-2Y | MEMC Singapore MEMC-M250ACA-20 | MEMC Singapore MEMC-M250ACC-20 | MEMC Singapore MEMC-M250ACC-21 | MEMC Singapore MEMC-M250AIC-20 | MEMC Singapore MEMC-M250AIC-21 | MEMC Singapore MEMC-M250AMA-20 | MEMC Singapore MEMC-M250AMC-20 | MEMC Singapore MEMC-M250AMC-21 | MEMC Singapore MEMC-M250LCA-20 | MEMC Singapore MEMC-M250LCC-20 | MEMC Singapore MEMC-M250LCC-21 | MEMC Singapore MEMC-M250LIC-20 | MEMC Singapore MEMC-M250LIC-21 | MEMC Singapore MEMC-M250LMA-20 | MEMC Singapore MEMC-M250LMC-20 | MEMC Singapore MEMC-M250LMC-21 | MEMC Singapore SE-M250KZC-2Y | MEMC Singapore MEMC-M255ACA-20 | MEMC Singapore MEMC-M255ACC-20 | MEMC Singapore MEMC-M255ACC-21 | MEMC Singapore MEMC-M255AIC-20 | MEMC Singapore MEMC-M255AIC-21 | MEMC Singapore MEMC-M255AMA-20 | MEMC Singapore MEMC-M255AMC-20 | MEMC Singapore MEMC-M255AMC-21 | MEMC Singapore MEMC-M255LCA-20 | MEMC Singapore MEMC-M255LCC-20 | MEMC Singapore MEMC-M255LCC-21 | MEMC Singapore MEMC-M255LIC-20 | MEMC Singapore MEMC-M255LIC-21 | MEMC Singapore MEMC-M255LMA-20 | MEMC Singapore MEMC-M255LMC-20 | MEMC Singapore MEMC-M255LMC-21 | MEMC Singapore SE-M255KZC-2Y | MEMC Singapore MEMC-M260ACA-20 | MEMC Singapore MEMC-M260ACC-20 | MEMC Singapore MEMC-M260ACC-21 | MEMC Singapore MEMC-M260AIC-20 | MEMC Singapore MEMC-M260AIC-21 | MEMC Singapore MEMC-M260AMA-20 | MEMC Singapore MEMC-M260AMC-20 | MEMC Singapore MEMC-M260AMC-21 | MEMC Singapore MEMC-M260LCA-20 | MEMC Singapore MEMC-M260LCC-20 | MEMC Singapore MEMC-M260LCC-21 | MEMC Singapore MEMC-M260LIC-20 | MEMC Singapore MEMC-M260LIC-21 | MEMC Singapore MEMC-M260LMA-20 | MEMC Singapore MEMC-M260LMC-20 | MEMC Singapore MEMC-M260LMC-21 | MEMC Singapore SE-M260KZC-2Y | MEMC Singapore MEMC-P270ACA | MEMC Singapore MEMC-P270ACC-21 | MEMC Singapore MEMC-P270ACC-25 | MEMC Singapore MEMC-P270ACC-26 | MEMC Singapore MEMC-P270AIC-20 | MEMC Singapore MEMC-P270AIC-24 | MEMC Singapore MEMC-P270AMA | MEMC Singapore MEMC-P270AMA-20 | MEMC Singapore MEMC-P270AMC-20 | MEMC Singapore MEMC-P270AMC-24 | MEMC Singapore MEMC-P270BCA-20 | MEMC Singapore MEMC-P270BCA-21 | MEMC Singapore MEMC-P270BCC-21 | MEMC Singapore MEMC-P270BCC-25 | MEMC Singapore MEMC-P270BCC-26 | MEMC Singapore MEMC-P270BCC-27 | MEMC Singapore MEMC-P270BMA-20 | MEMC Singapore MEMC-P270BMC-20 | MEMC Singapore MEMC-P270BMC-24 | MEMC Singapore MEMC-P270BMC-25 | MEMC Singapore MEMC-P270BMC-26 | MEMC Singapore MEMC-P270BMC-27 | MEMC Singapore MEMC-M275ACA-20 | MEMC Singapore MEMC-M275ACA-21 | MEMC Singapore MEMC-M275AMA-20 | MEMC Singapore MEMC-M275BCA-20 | MEMC Singapore MEMC-M275BCA-21 | MEMC Singapore MEMC-M275BMA-20 | MEMC Singapore MEMC-P275ACA | MEMC Singapore MEMC-P275ACA-20 | MEMC Singapore MEMC-P275ACA-21 | MEMC Singapore MEMC-P275ACC-21 | MEMC Singapore MEMC-P275ACC-25 | MEMC Singapore MEMC-P275ACC-26 | MEMC Singapore MEMC-P275AIC-20 | MEMC Singapore MEMC-P275AIC-24 | MEMC Singapore MEMC-P275AMA | MEMC Singapore MEMC-P275AMA-20 | MEMC Singapore MEMC-P275AMC-20 | MEMC Singapore MEMC-P275AMC-24 | MEMC Singapore MEMC-P275BCA-20 | MEMC Singapore MEMC-P275BCA-21 | MEMC Singapore MEMC-P275BCC-21 | MEMC Singapore MEMC-P275BCC-25 | MEMC Singapore MEMC-P275BCC-26 | MEMC Singapore MEMC-P275BCC-27 | MEMC Singapore MEMC-P275BMA-20 | MEMC Singapore MEMC-P275BMC-20 | MEMC Singapore MEMC-P275BMC-24 | MEMC Singapore MEMC-P275BMC-25 | MEMC Singapore MEMC-P275BMC-26 | MEMC Singapore MEMC-P275BMC-27 | MEMC Singapore MEMC-M280ACA-20 | MEMC Singapore MEMC-M280ACA-21 | MEMC Singapore MEMC-M280AMA-20 | MEMC Singapore MEMC-M280BCA-20 | MEMC Singapore MEMC-M280BCA-21 | MEMC Singapore MEMC-M280BMA-20 | MEMC Singapore MEMC-P280ACA | MEMC Singapore MEMC-P280ACA-20 | MEMC Singapore MEMC-P280ACA-21 | MEMC Singapore MEMC-P280ACC-21 | MEMC Singapore MEMC-P280ACC-25 | MEMC Singapore MEMC-P280ACC-26 | MEMC Singapore MEMC-P280AIC-20 | MEMC Singapore MEMC-P280AIC-24 | MEMC Singapore MEMC-P280AMA | MEMC Singapore MEMC-P280AMA-20 | MEMC Singapore MEMC-P280AMC-20 | MEMC Singapore MEMC-P280AMC-24 | MEMC Singapore MEMC-P280BCA-20 | MEMC Singapore MEMC-P280BCA-21 | MEMC Singapore MEMC-P280BCC-21 | MEMC Singapore MEMC-P280BCC-25 | MEMC Singapore MEMC-P280BCC-26 | MEMC Singapore MEMC-P280BCC-27 | MEMC Singapore MEMC-P280BMA-20 | MEMC Singapore MEMC-P280BMC-20 | MEMC Singapore MEMC-P280BMC-24 | MEMC Singapore MEMC-P280BMC-25 | MEMC Singapore MEMC-P280BMC-26 | MEMC Singapore MEMC-P280BMC-27 | MEMC Singapore MEMC-P280BZC-3Y | MEMC Singapore MEMC-M285ACA-20 | MEMC Singapore MEMC-M285ACA-21 | MEMC Singapore MEMC-M285AMA-20 | MEMC Singapore MEMC-M285BCA-20 | MEMC Singapore MEMC-M285BCA-21 | MEMC Singapore MEMC-M285BMA-20 | MEMC Singapore MEMC-P285ACA | MEMC Singapore MEMC-P285ACA-20 | MEMC Singapore MEMC-P285ACA-21 | MEMC Singapore MEMC-P285ACC-21 | MEMC Singapore MEMC-P285ACC-25 | MEMC Singapore MEMC-P285ACC-26 | MEMC Singapore MEMC-P285AIC-20 | MEMC Singapore MEMC-P285AIC-24 | MEMC Singapore MEMC-P285AMA | MEMC Singapore MEMC-P285AMA-20 | MEMC Singapore MEMC-P285AMC-20 | MEMC Singapore MEMC-P285AMC-24 | MEMC Singapore MEMC-P285BCA-20 | MEMC Singapore MEMC-P285BCA-21 | MEMC Singapore MEMC-P285BCC-21 | MEMC Singapore MEMC-P285BCC-25 | MEMC Singapore MEMC-P285BCC-26 | MEMC Singapore MEMC-P285BCC-27 | MEMC Singapore MEMC-P285BMA-20 | MEMC Singapore MEMC-P285BMC-20 | MEMC Singapore MEMC-P285BMC-24 | MEMC Singapore MEMC-P285BMC-25 | MEMC Singapore MEMC-P285BMC-26 | MEMC Singapore MEMC-P285BMC-27 | MEMC Singapore MEMC-P285BZC-3Y | MEMC Singapore MEMC-M290ACA-20 | MEMC Singapore MEMC-M290ACA-21 | MEMC Singapore MEMC-M290ACC-24 | MEMC Singapore MEMC-M290ACC-27 | MEMC Singapore MEMC-M290AEC-24 | MEMC Singapore MEMC-M290AEC-27 | MEMC Singapore MEMC-M290AMA-20 | MEMC Singapore MEMC-M290AMC-24 | MEMC Singapore MEMC-M290AMC-27 | MEMC Singapore MEMC-M290BCA-20 | MEMC Singapore MEMC-M290BCA-21 | MEMC Singapore MEMC-M290BCC-24 | MEMC Singapore MEMC-M290BCC-27 | MEMC Singapore MEMC-M290BEC-24 | MEMC Singapore MEMC-M290BEC-27 | MEMC Singapore MEMC-M290BMA-20 | MEMC Singapore MEMC-M290BMC-24 | MEMC Singapore MEMC-M290BMC-27 | MEMC Singapore MEMC-P290ACA | MEMC Singapore MEMC-P290ACA-20 | MEMC Singapore MEMC-P290ACA-21 | MEMC Singapore MEMC-P290ACC-21 | MEMC Singapore MEMC-P290ACC-25 | MEMC Singapore MEMC-P290ACC-26 | MEMC Singapore MEMC-P290AIC-20 | MEMC Singapore MEMC-P290AIC-24 | MEMC Singapore MEMC-P290AMA | MEMC Singapore MEMC-P290AMA-20 | MEMC Singapore MEMC-P290AMC-20 | MEMC Singapore MEMC-P290AMC-24 | MEMC Singapore MEMC-P290BCA-20 | MEMC Singapore MEMC-P290BCA-21 | MEMC Singapore MEMC-P290BCC-21 | MEMC Singapore MEMC-P290BCC-25 | MEMC Singapore MEMC-P290BCC-26 | MEMC Singapore MEMC-P290BCC-27 | MEMC Singapore MEMC-P290BMA-20 | MEMC Singapore MEMC-P290BMC-20 | MEMC Singapore MEMC-P290BMC-24 | MEMC Singapore MEMC-P290BMC-25 | MEMC Singapore MEMC-P290BMC-26 | MEMC Singapore MEMC-P290BMC-27 | MEMC Singapore MEMC-P290BZC-3Y | MEMC Singapore MEMC-Q290ACC-34 | MEMC Singapore MEMC-Q290ACC-35 | MEMC Singapore MEMC-Q290ACC-36 | MEMC Singapore MEMC-Q290AEC-34 | MEMC Singapore MEMC-Q290AEC-35 | MEMC Singapore MEMC-Q290AEC-36 | MEMC Singapore MEMC-Q290AMC-34 | MEMC Singapore MEMC-Q290AMC-35 | MEMC Singapore MEMC-Q290AMC-36 | MEMC Singapore MEMC-Q290BZC-3Y | MEMC Singapore SE-M290BZC-3Y | MEMC Singapore MEMC-M295ACA-20 | MEMC Singapore MEMC-M295ACA-21 | MEMC Singapore MEMC-M295ACC-24 | MEMC Singapore MEMC-M295ACC-27 | MEMC Singapore MEMC-M295AEC-24 | MEMC Singapore MEMC-M295AEC-27 | MEMC Singapore MEMC-M295AMA-20 | MEMC Singapore MEMC-M295AMC-24 | MEMC Singapore MEMC-M295AMC-27 | MEMC Singapore MEMC-M295BCA-20 | MEMC Singapore MEMC-M295BCA-21 | MEMC Singapore MEMC-M295BCC-24 | MEMC Singapore MEMC-M295BCC-27 | MEMC Singapore MEMC-M295BEC-24 | MEMC Singapore MEMC-M295BEC-27 | MEMC Singapore MEMC-M295BMA-20 | MEMC Singapore MEMC-M295BMC-24 | MEMC Singapore MEMC-M295BMC-27 | MEMC Singapore MEMC-P295ACC-21 | MEMC Singapore MEMC-P295ACC-25 | MEMC Singapore MEMC-P295ACC-26 | MEMC Singapore MEMC-P295AIC-20 | MEMC Singapore MEMC-P295AIC-24 | MEMC Singapore MEMC-P295AMC-20 | MEMC Singapore MEMC-P295AMC-24 | MEMC Singapore MEMC-P295BCC-21 | MEMC Singapore MEMC-P295BCC-25 | MEMC Singapore MEMC-P295BCC-26 | MEMC Singapore MEMC-P295BCC-27 | MEMC Singapore MEMC-P295BMC-20 | MEMC Singapore MEMC-P295BMC-24 | MEMC Singapore MEMC-P295BMC-25 | MEMC Singapore MEMC-P295BMC-26 | MEMC Singapore MEMC-P295BMC-27 | MEMC Singapore MEMC-P295BZC-3Y | MEMC Singapore MEMC-Q295ACC-34 | MEMC Singapore MEMC-Q295ACC-35 | MEMC Singapore MEMC-Q295ACC-36 | MEMC Singapore MEMC-Q295AEC-34 | MEMC Singapore MEMC-Q295AEC-35 | MEMC Singapore MEMC-Q295AEC-36 | MEMC Singapore MEMC-Q295AMC-34 | MEMC Singapore MEMC-Q295AMC-35 | MEMC Singapore MEMC-Q295AMC-36 | MEMC Singapore MEMC-Q295BZC-3Y | MEMC Singapore SE-M295BZC-3Y | MEMC Singapore MEMC-M300ACC-24 | MEMC Singapore MEMC-M300ACC-27 | MEMC Singapore MEMC-M300AEC-24 | MEMC Singapore MEMC-M300AEC-27 | MEMC Singapore MEMC-M300AMC-24 | MEMC Singapore MEMC-M300AMC-27 | MEMC Singapore MEMC-M300BCC-24 | MEMC Singapore MEMC-M300BCC-27 | MEMC Singapore MEMC-M300BEC-24 | MEMC Singapore MEMC-M300BEC-27 | MEMC Singapore MEMC-M300BMC-24 | MEMC Singapore MEMC-M300BMC-27 | MEMC Singapore MEMC-M300BZC-3Y | MEMC Singapore MEMC-P300BCC-21 | MEMC Singapore MEMC-P300BCC-25 | MEMC Singapore MEMC-P300BCC-26 | MEMC Singapore MEMC-P300BCC-27 | MEMC Singapore MEMC-P300BMC-20 | MEMC Singapore MEMC-P300BMC-24 | MEMC Singapore MEMC-P300BMC-25 | MEMC Singapore MEMC-P300BMC-26 | MEMC Singapore MEMC-P300BMC-27 | MEMC Singapore MEMC-P300BZC-3Y | MEMC Singapore MEMC-Q300ACC-34 | MEMC Singapore MEMC-Q300ACC-35 | MEMC Singapore MEMC-Q300ACC-36 | MEMC Singapore MEMC-Q300AEC-34 | MEMC Singapore MEMC-Q300AEC-35 | MEMC Singapore MEMC-Q300AEC-36 | MEMC Singapore MEMC-Q300AMC-34 | MEMC Singapore MEMC-Q300AMC-35 | MEMC Singapore MEMC-Q300AMC-36 | MEMC Singapore MEMC-Q300BZC-3Y | MEMC Singapore SE-M300BZC-3Y | MEMC Singapore MEMC-M305ACC-24 | MEMC Singapore MEMC-M305ACC-27 | MEMC Singapore MEMC-M305AEC-24 | MEMC Singapore MEMC-M305AEC-27 | MEMC Singapore MEMC-M305AMC-24 | MEMC Singapore MEMC-M305AMC-27 | MEMC Singapore MEMC-M305BCC-24 | MEMC Singapore MEMC-M305BCC-27 | MEMC Singapore MEMC-M305BEC-24 | MEMC Singapore MEMC-M305BEC-27 | MEMC Singapore MEMC-M305BMC-24 | MEMC Singapore MEMC-M305BMC-27 | MEMC Singapore MEMC-M305BZC-3Y | MEMC Singapore MEMC-P305BCC-21 | MEMC Singapore MEMC-P305BCC-25 | MEMC Singapore MEMC-P305BCC-26 | MEMC Singapore MEMC-P305BCC-27 | MEMC Singapore MEMC-P305BMC-20 | MEMC Singapore MEMC-P305BMC-24 | MEMC Singapore MEMC-P305BMC-25 | MEMC Singapore MEMC-P305BMC-26 | MEMC Singapore MEMC-P305BMC-27 | MEMC Singapore MEMC-P305BZC-3Y | MEMC Singapore MEMC-Q305ACC-34 | MEMC Singapore MEMC-Q305ACC-35 | MEMC Singapore MEMC-Q305ACC-36 | MEMC Singapore MEMC-Q305AEC-34 | MEMC Singapore MEMC-Q305AEC-35 | MEMC Singapore MEMC-Q305AEC-36 | MEMC Singapore MEMC-Q305AMC-34 | MEMC Singapore MEMC-Q305AMC-35 | MEMC Singapore MEMC-Q305AMC-36 | MEMC Singapore MEMC-Q305BZC-3Y | MEMC Singapore SE-M305BZC-3Y | MEMC Singapore MEMC-M310BZC-3Y | MEMC Singapore MEMC-Q310ACC-34 | MEMC Singapore MEMC-Q310ACC-35 | MEMC Singapore MEMC-Q310ACC-36 | MEMC Singapore MEMC-Q310AEC-34 | MEMC Singapore MEMC-Q310AEC-35 | MEMC Singapore MEMC-Q310AEC-36 | MEMC Singapore MEMC-Q310AMC-34 | MEMC Singapore MEMC-Q310AMC-35 | MEMC Singapore MEMC-Q310AMC-36 | MEMC Singapore MEMC-Q310BZC-3Y | MEMC Singapore SE-F310BZC-3Y | MEMC Singapore SE-M310BZC-3Y | MEMC Singapore MEMC-M315BZC-3Y | MEMC Singapore MEMC-Q315ACC-34 | MEMC Singapore MEMC-Q315ACC-35 | MEMC Singapore MEMC-Q315ACC-36 | MEMC Singapore MEMC-Q315AEC-34 | MEMC Singapore MEMC-Q315AEC-35 | MEMC Singapore MEMC-Q315AEC-36 | MEMC Singapore MEMC-Q315AMC-34 | MEMC Singapore MEMC-Q315AMC-35 | MEMC Singapore MEMC-Q315AMC-36 | MEMC Singapore MEMC-Q315BZC-3Y | MEMC Singapore SE-F315BZC-3Y | MEMC Singapore SE-M315BZC-3Y | MEMC Singapore MEMC-M320BZC-3Y | MEMC Singapore MEMC-Q320ACC-34 | MEMC Singapore MEMC-Q320ACC-35 | MEMC Singapore MEMC-Q320ACC-36 | MEMC Singapore MEMC-Q320AEC-34 | MEMC Singapore MEMC-Q320AEC-35 | MEMC Singapore MEMC-Q320AEC-36 | MEMC Singapore MEMC-Q320AMC-34 | MEMC Singapore MEMC-Q320AMC-35 | MEMC Singapore MEMC-Q320AMC-36 | MEMC Singapore MEMC-Q320BZC-3Y | MEMC Singapore SE-F320BZC-3Y | MEMC Singapore SE-M320BZC-3Y | MEMC Singapore MEMC-M325BZC-3Y | MEMC Singapore SE-F325BZC-3Y | MEMC Singapore MEMC-M330BZC-3Y | MEMC Singapore SE-F330BZC-3Y | MEMC Singapore SE-F335BZC-3Y | Mitsubishi Electric PV-EE120MF5F | Mitsubishi Electric PV-EE125MF5F | Mitsubishi Electric PV-EE130MF5F | Mitsubishi Electric PV-MF160EB4 | Mitsubishi Electric PV-MF165EB4 | Mitsubishi Electric PV-MF170EB3 | Mitsubishi Electric PV-MF170EB4 | Mitsubishi Electric PV-MF170UD4 | Mitsubishi Electric PV-UD170MF5 | Mitsubishi Electric PV-MF175UD4 | Mitsubishi Electric PV-UD175MF5 | Mitsubishi Electric PV-MF180UD4 | Mitsubishi Electric PV-UD180MF5 | Mitsubishi Electric PV-UD185HA6 | Mitsubishi Electric PV-UD185MF5 | Mitsubishi Electric PV-UD190HA6 | Mitsubishi Electric PV-UD190MF5 | Mitsubishi Electric PV-UD195HA6 | Mitsubishi Electric PV-UJ212G6 | Mitsubishi Electric PV-UJ218G6 | Mitsubishi Electric PV-UJ220GA6 | Mitsubishi Electric PV-UJ220GA6-D | Mitsubishi Electric PV-UJ224G6 | Mitsubishi Electric PV-UJ225GA6 | Mitsubishi Electric PV-UJ225GA6-D | Mitsubishi Electric PV-UJ230GA6 | Mitsubishi Electric PV-UJ230GA6-D | Mitsubishi Electric PV-MJU235GB | Mitsubishi Electric PV-UJ235GA6 | Mitsubishi Electric PV-UJ235GA6-D | Mitsubishi Electric PV-MJU240GB | Mitsubishi Electric PV-MJU245GB | Mitsubishi Electric PV-MLU250HC | Mitsubishi Electric PV-MLE255HD | Mitsubishi Electric PV-MLU255HC | Mitsubishi Electric PV-MLE260HD | Mitsubishi Electric PV-MLU260HC | Montech Solar MTS-215-P | Montech Solar MTS-220-P | Montech Solar MTS-225-P | Montech Solar MTS-230-P | Montech Solar MTS-235-M | Montech Solar MTS-240-M | Montech Solar MTS-245-M | Montech Solar MTS-250-M | Moser Baer Photovoltaic MBPV CAAP 210 | Moser Baer Photovoltaic MBPV CAAP BB 210W | Moser Baer Photovoltaic MBPV CAAP 215W | Moser Baer Photovoltaic MBPV CAAP BB 215W | Moser Baer Photovoltaic MBPV CAAP 220 | Moser Baer Photovoltaic MBPV CAAP BB 220W | Moser Baer Photovoltaic MBPV CAAP BB 225W | Moser Baer Photovoltaic MBPV CAAP BB 230W | Moser Baer Photovoltaic MBPV CAAP BB 235W | Moser Baer Photovoltaic MBPV CAAP BB 240W | Moser Baer Photovoltaic MBPV CAAP BB 245W | Moser Baer Solar MBSL eLITE 60 3x 225 | Moser Baer Solar MBSL eLITE 60 3x 230 | Moser Baer Solar MBSL eLITE 60 3x 235 | Moser Baer Solar MBSL eLITE 60 3x 240 | Moser Baer Solar MBSL eLITE 60 3x 245 | Motech Americas IM54B2-200-XXXXXX | Motech Americas IM54C2-200-XXXXXX | Motech Americas IM54C3-200-XXXXXX | Motech Americas IM54D2-200-XXXXXX | Motech Americas IM54D3-200-XXXXXX | Motech Americas GEPVp-205-MSA | Motech Americas GEPVp-205-MSB | Motech Americas IM54B2-205-XXXXXX | Motech Americas IM54B3-205-XXXXXX | Motech Americas IM54C2-205-XXXXXX | Motech Americas IM54C3-205-XXXXXX | Motech Americas IM54D2-205-XXXXXX | Motech Americas IM54D3-205-XXXXXX | Motech Americas GEPVp-210-MSA | Motech Americas GEPVp-210-MSB | Motech Americas IM54B2-210-XXXXXX | Motech Americas IM54B3-210-XXXXXX | Motech Americas IM54C2-210-XXXXXX | Motech Americas IM54C3-210-XXXXXX | Motech Americas IM54D2-210-XXXXXX | Motech Americas IM54D3-210-XXXXXX | Motech Americas XS54B3-210-XXXXXX | Motech Americas XS54C3-210-XXXXXX | Motech Americas XS54D3-210-XXXXXX | Motech Americas IM54B2-215-XXXXXX | Motech Americas IM54B3-215-XXXXXX | Motech Americas IM54C2-215-XXXXXX | Motech Americas IM54C3-215-XXXXXX | Motech Americas IM54D2-215-XXXXXX | Motech Americas IM54D3-215-XXXXXX | Motech Americas XS54B3-215-XXXXXX | Motech Americas XS54C3-215-XXXXXX | Motech Americas XS54D3-215-XXXXXX | Motech Americas IM54B3-220-XXXXXX | Motech Americas IM54C2-220-XXXXXX | Motech Americas IM54C3-220-XXXXXX | Motech Americas IM54D2-220-XXXXXX | Motech Americas IM54D3-220-XXXXXX | Motech Americas XS54B3-220-XXXXXX | Motech Americas XS54C3-220-XXXXXX | Motech Americas XS54D3-220-XXXXXX | Motech Americas IM54B3-225-XXXXXX | Motech Americas IM54C3-225-XXXXXX | Motech Americas IM54D3-225-XXXXXX | Motech Americas IM60B2-225-XXXXXX | Motech Americas IM60B3-225-XXXXXX | Motech Americas XS54B3-225-XXXXXX | Motech Americas XS54C3-225-XXXXXX | Motech Americas XS54D3-225-XXXXXX | Motech Americas IM60B2-230-XXXXXX | Motech Americas IM60B3-230-XXXXXX | Motech Americas IM60C3-230-XXXXXX | Motech Americas IM60D3-230-XXXXXX | Motech Americas MTPVp-230-MSB | Motech Americas MTPVp-230-MSC | Motech Americas MTPVp-230-MSD | Motech Americas XS54B3-230-XXXXXX | Motech Americas XS54C3-230-XXXXXX | Motech Americas XS54D3-230-XXXXXX | Motech Americas IM60B2-235-XXXXXX | Motech Americas IM60B3-235-XXXXXX | Motech Americas IM60C2-235-XXXXXX | Motech Americas IM60C3-235-XXXXXX | Motech Americas IM60D2-235-XXXXXX | Motech Americas IM60D3-235-XXXXXX | Motech Americas MTPVp-235-MSB | Motech Americas MTPVp-235-MSC | Motech Americas MTPVp-235-MSD | Motech Americas XS54C3-235-XXXXXX | Motech Americas XS60B3-235-XXXXXX | Motech Americas XS60C3-235-XXXXXX | Motech Americas XS60D3-235-XXXXXX | Motech Americas IM60B2-240-XXXXXX | Motech Americas IM60B3-240-XXXXXX | Motech Americas IM60C2-240-XXXXXX | Motech Americas IM60C3-240-XXXXXX | Motech Americas IM60D2-240-XXXXXX | Motech Americas IM60D3-240-XXXXXX | Motech Americas MTPVp-240-MSB | Motech Americas MTPVp-240-MSC | Motech Americas MTPVp-240-MSD | Motech Americas XS60B3-240-XXXXXX | Motech Americas XS60C3-240-XXXXXX | Motech Americas XS60D3-240-XXXXXX | Motech Americas IM60B2-245-XXXXXX | Motech Americas IM60B3-245-XXXXXX | Motech Americas IM60C2-245-XXXXXX | Motech Americas IM60C3-245-XXXXXX | Motech Americas IM60D2-245-XXXXXX | Motech Americas IM60D3-245-XXXXXX | Motech Americas MTPVp-245-MSB | Motech Americas MTPVp-245-MSC | Motech Americas MTPVp-245-MSD | Motech Americas XS60B3-245-XXXXXX | Motech Americas XS60C3-245-XXXXXX | Motech Americas XS60D3-245-XXXXXX | Motech Americas IM60B3-250-XXXXXX | Motech Americas IM60C2-250-XXXXXX | Motech Americas IM60C3-250-XXXXXX | Motech Americas IM60D2-250-XXXXXX | Motech Americas IM60D3-250-XXXXXX | Motech Americas XS60B3-250-XXXXXX | Motech Americas XS60C3-250-XXXXXX | Motech Americas XS60D3-250-XXXXXX | Motech Americas IM60B3-255-XXXXXX | Motech Americas IM60C3-255-XXXXXX | Motech Americas IM60D3-255-XXXXXX | Motech Americas XS60B3-255-XXXXXX | Motech Americas XS60C3-255-XXXXXX | Motech Americas XS60D3-255-XXXXXX | Motech Americas IM60B3-260-XXXXXX | Motech Americas IM60C3-260-XXXXXX | Motech Americas IM60D3-260-XXXXXX | Motech Americas XS60B3-260-XXXXXX | Motech Americas XS60C3-260-XXXXXX | Motech Americas XS60D3-260-XXXXXX | Motech Americas IM60B3-265-XXXXXX | Motech Americas IM60C3-265-XXXXXX | Motech Americas IM60D3-265-XXXXXX | Motech Americas XS60B3-265-XXXXXX | Motech Americas XS60C3-265-XXXXXX | Motech Americas XS60D3-265-XXXXXX | Motech Americas IM60B3-270-XXXXXX | Motech Americas IM60C3-270-XXXXXX | Motech Americas IM60D3-270-XXXXXX | Motech Americas XS60C3-270-XXXXXX | Motech Americas XS60D3-270-XXXXXX | Motech Americas IM72C2-280-XXXXXX | Motech Americas IM72C3-280-XXXXXX | Motech Americas IM72D2-280-XXXXXX | Motech Americas IM72D3-280-XXXXXX | Motech Americas MTPVp-280-MSC | Motech Americas IM72C2-285-XXXXXX | Motech Americas IM72C3-285-XXXXXX | Motech Americas IM72D2-285-XXXXXX | Motech Americas IM72D3-285-XXXXXX | Motech Americas MTPVp-285-MSC | Motech Americas XS72C3-285-XXXXXX | Motech Americas XS72D3-285-XXXXXX | Motech Americas IM72C2-290-XXXXXX | Motech Americas IM72C3-290-XXXXXX | Motech Americas IM72D2-290-XXXXXX | Motech Americas IM72D3-290-XXXXXX | Motech Americas MTPVp-290-MSC | Motech Americas XS72C3-290-XXXXXX | Motech Americas XS72D3-290-XXXXXX | Motech Americas IM72C2-295-XXXXXX | Motech Americas IM72C3-295-XXXXXX | Motech Americas IM72D2-295-XXXXXX | Motech Americas IM72D3-295-XXXXXX | Motech Americas MTPVp-295-MSC | Motech Americas XS72C3-295-XXXXXX | Motech Americas XS72D3-295-XXXXXX | Motech Americas IM72C3-300-XXXXXX | Motech Americas IM72D3-300-XXXXXX | Motech Americas XS72C3-300-XXXXXX | Motech Americas XS72D3-300-XXXXXX | Motech Americas IM72C3-305-XXXXXX | Motech Americas IM72D3-305-XXXXXX | Motech Americas XS72C3-305-XXXXXX | Motech Americas XS72D3-305-XXXXXX | Motech Americas IM72C3-310-XXXXXX | Motech Americas IM72D3-310-XXXXXX | Motech Americas XS72C3-310-XXXXXX | Motech Americas XS72D3-310-XXXXXX | Motech Americas IM72C3-315-XXXXXX | Motech Americas IM72D3-315-XXXXXX | Motech Americas XS72C3-315-XXXXXX | Motech Americas XS72D3-315-XXXXXX | Motech Americas IM72C3-320-XXXXXX | Motech Americas IM72D3-320-XXXXXX | Motech Americas XS72C3-320-XXXXXX | Motech Americas XS72D3-320-XXXXXX | Motech Americas IM72C3-325-XXXXXX | Motech Americas IM72D3-325-XXXXXX | Motech Americas XS72C3-325-XXXXXX | Motech Americas XS72D3-325-XXXXXX | Motech Americas IM72C3-330-XXXXXX | Motech Americas IM72D3-330-XXXXXX | Motech Americas XS72C3-330-XXXXXX | Motech Americas XS72D3-330-XXXXXX | MX Solar USA MX60-220 | MX Solar USA MX60-225 | MX Solar USA MX60-230 | MX Solar USA MX60-235 | MX Solar USA MX60-240 | MX Solar USA MX60-245 | Nanjing Daqo New Energy DQ180MFAb | Nanjing Daqo New Energy DQ185MFAb | Nanjing Daqo New Energy DQ190MFAb | Nanjing Daqo New Energy DQ190PSBb | Nanjing Daqo New Energy DQ195PSBb | Nanjing Daqo New Energy DQ200PSBb | Nanjing Daqo New Energy DQ205PSBb | Nanjing Daqo New Energy DQ210PSBb | Nanjing Daqo New Energy DQ220PSCb | Nanjing Daqo New Energy DQ225PSCb | Nanjing Daqo New Energy DQ230PSCb | Nanjing Daqo New Energy DQ235PSCb | Nanjing Daqo New Energy DQ240PSCb | Nanosolar Nanosolar Utility Panel 200W | Nantong Qiangsheng Photovoltaic Technology QS85EGF | Nantong Qiangsheng Photovoltaic Technology QS90EGF | Neo Solar Power D6P120A1F | Neo Solar Power D6P125A1F | Neo Solar Power D6P130A1F | Neo Solar Power D6P135A1F | Neo Solar Power D6P140A1F | Neo Solar Power D6P190A5F | Neo Solar Power D6P195A5F | Neo Solar Power D6P200A5F | Neo Solar Power D6P205A5F | Neo Solar Power D6P210A5F | Neo Solar Power D6P215A3F | Neo Solar Power D6P215A5F | Neo Solar Power D6P220A3F | Neo Solar Power D6P220A5F | Neo Solar Power 7C00-6A225 | Neo Solar Power 7C00-6A225-B | Neo Solar Power D6P225A3F | Neo Solar Power 7C00-6A230 | Neo Solar Power 7C00-6A230-B | Neo Solar Power D6P230A3F | Neo Solar Power D6P230B3A | Neo Solar Power 7C00-6A235 | Neo Solar Power 7C00-6A235-B | Neo Solar Power 7E00-6A235 | Neo Solar Power 7E00-6A235-B | Neo Solar Power D6M235B3A | Neo Solar Power D6P235A3F | Neo Solar Power D6P235B3A | Neo Solar Power 7C00-6A240 | Neo Solar Power 7C00-6A240-B | Neo Solar Power 7E00-6A240 | Neo Solar Power 7E00-6A240-B | Neo Solar Power D6M240B3A | Neo Solar Power D6P240A3F | Neo Solar Power D6P240B3A | Neo Solar Power 7C00-6A245 | Neo Solar Power 7C00-6A245-B | Neo Solar Power 7E00-6A245 | Neo Solar Power 7E00-6A245-B | Neo Solar Power D6M245B3A | Neo Solar Power D6P245A3F | Neo Solar Power D6P245B3A | Neo Solar Power 7E00-6A250 | Neo Solar Power 7E00-6A250-B | Neo Solar Power D6M250B3A | Neo Solar Power D6P250B3A | Neo Solar Power 7E00-6A255 | Neo Solar Power 7E00-6A255-B | Neo Solar Power D6M255B3A | Neo Solar Power 7E00-6A260 | Neo Solar Power 7E00-6A260-B | Neo Solar Power D6P260A4F | Neo Solar Power 7E00-6A265 | Neo Solar Power 7E00-6A265-B | Neo Solar Power D6P265A4F | Neo Solar Power D6P270A4F | Neo Solar Power 7C00-6C275 | Neo Solar Power 7C00-6C275-B | Neo Solar Power D6P275A4F | Neo Solar Power D6P275B4A | Neo Solar Power D6Q275B4A | Neo Solar Power 7C00-6C280 | Neo Solar Power 7C00-6C280-B | Neo Solar Power D6P280A4F | Neo Solar Power D6P280B4A | Neo Solar Power D6Q280B4A | Neo Solar Power 7C00-6C285 | Neo Solar Power 7C00-6C285-B | Neo Solar Power 7E00-6C285 | Neo Solar Power 7E00-6C285-B | Neo Solar Power D6M285B4A | Neo Solar Power D6P285A4F | Neo Solar Power D6P285B4A | Neo Solar Power D6Q285B4A | Neo Solar Power 7C00-6C290 | Neo Solar Power 7C00-6C290-B | Neo Solar Power 7E00-6C290 | Neo Solar Power 7E00-6C290-B | Neo Solar Power D6M290B4A | Neo Solar Power D6P290A4F | Neo Solar Power D6P290B4A | Neo Solar Power D6Q290B4A | Neo Solar Power 7C00-6C295 | Neo Solar Power 7C00-6C295-B | Neo Solar Power 7E00-6C295 | Neo Solar Power 7E00-6C295-B | Neo Solar Power D6M295B4A | Neo Solar Power D6P295B4A | Neo Solar Power D6Q295B4A | Neo Solar Power 7E00-6C300 | Neo Solar Power 7E00-6C300-B | Neo Solar Power D6M300B4A | Neo Solar Power 7E00-6C305 | Neo Solar Power 7E00-6C305-B | Neo Solar Power D6M305B4A | Nexpower Technology NH-100UT_3A | NexPower Technology NH-100UX 3A | Nexpower Technology NH-100UT_4A | NexPower Technology NH-100UX 4A | Nexpower Technology NH-100UT_5A | NexPower Technology NH-100UX 5A | Nexpower Technology NH-100UT_6A | Nexpower Technology NT-125UX | Nexpower Technology NT-130UX | Nexpower Technology NT-135UX | NexPower Technology NT-140UX | NexPower Technology NT-145UX | NexPower Technology NT-150 | NexPower Technology NT-155 | NexPower Technology NT-160 | Next Solar Systems NXT18m | Next Solar Systems NXT20e | NICOR NS-H115M54-01 | NICOR NS-H120M54-01 | NICOR NS-H125M54-01 | NICOR NS-H160M72-01 | NICOR NS-H165M72-01 | NICOR NS-H170M72-01 | NICOR NS-H175M72-01 | NICOR NS-H180M72-01 | NICOR NS-H185M72-01 | NICOR NS-H190M72-01 | NICOR NS-H195M72-01 | NICOR NS-H200M72-01 | NICOR NS-H200P60-01 | NICOR NS-H205P60-01 | NICOR NS-H210P60-01 | NICOR NS-H215P60-01 | NICOR NS-H220P60-01 | NICOR NS-H225P60-01 | NICOR NS-H230P60-01 | NICOR NS-H235P60-01 | NICOR NS-H240P60-01 | Ningbo Best Solar Energy Technology B155(35)P1580X800 | Ningbo Best Solar Energy Technology B160(35)P1580X800 | Ningbo Best Solar Energy Technology B165(35)P1580X800 | Ningbo Best Solar Energy Technology B175(35)P1580X800 | Ningbo Best Solar Energy Technology B180(35)P1580X800 | Ningbo Maxsolar MP-150WP | Ningbo Maxsolar MP-155WP | Ningbo Maxsolar MP-160WP | Ningbo Maxsolar MP-165WP | Ningbo Maxsolar MP-170WP | Ningbo Maxsolar MP-175WP | Ningbo Maxsolar MP-180WP | Ningbo Qixin Solar Electrical Appliance SL160UL-36M | Ningbo Qixin Solar Electrical Appliance SL165UL-36M | Ningbo Qixin Solar Electrical Appliance SL170UL-36M | Ningbo Qixin Solar Electrical Appliance SL180UL-36M | Ningbo Qixin Solar Electrical Appliance SL185UL-36M | Ningbo Qixin Solar Electrical Appliance SL210UL-30P | Ningbo Qixin Solar Electrical Appliance SL215UL-30P | Ningbo Qixin Solar Electrical Appliance SL220UL-30P | Ningbo Qixin Solar Electrical Appliance SL220UL-48M | Ningbo Qixin Solar Electrical Appliance SL225UL-30P | Ningbo Qixin Solar Electrical Appliance SL225UL-48M | Ningbo Qixin Solar Electrical Appliance SL230UL-30P | Ningbo Qixin Solar Electrical Appliance SL230UL-48M | Ningbo Qixin Solar Electrical Appliance SL235UL-30P | Ningbo Qixin Solar Electrical Appliance SL235UL-48M | Ningbo Qixin Solar Electrical Appliance SL240UL-48M | Ningbo Qixin Solar Electrical Appliance SL245UL-48M | Ningbo Qixin Solar Electrical Appliance SL250UL-36M | Ningbo Qixin Solar Electrical Appliance SL250UL-48M | Ningbo Qixin Solar Electrical Appliance SL255UL-36M | Ningbo Qixin Solar Electrical Appliance SL260UL-36M | Ningbo Qixin Solar Electrical Appliance SL265UL-36M | Ningbo Qixin Solar Electrical Appliance SL270UL-36M | Ningbo Qixin Solar Electrical Appliance SL275UL-36M | Ningbo Qixin Solar Electrical Appliance SL280UL-36M | Ningbo Solar Electric Power TDB125x125-72-P 150W | Ningbo Solar Electric Power TPB125x125-72-P 150W | Ningbo Solar Electric Power TDB125x125-72-P 155W | Ningbo Solar Electric Power TPB125x125-72-P 155W | Ningbo Solar Electric Power TDB125x125-72-P 160W | Ningbo Solar Electric Power TPB125x125-72-P 160W | Ningbo Solar Electric Power TDB125x125-72-P 165W | Ningbo Solar Electric Power TPB125x125-72-P 165W | Ningbo Solar Electric Power TDB125x125-72-P 170W | Ningbo Solar Electric Power TPB125x125-72-P 170W | Ningbo Solar Electric Power TDB125x125-72-P 175W | Ningbo Solar Electric Power TPB125x125-72-P 175W | Ningbo Solar Electric Power TDB125x125-72-P 180W | Ningbo Solar Electric Power TPB125x125-72-P 180W | Ningbo Solar Electric Power TPB156x156-54-P 180W | Ningbo Solar Electric Power TPB156x156-54-P 185W | Ningbo Solar Electric Power TPB156x156-54-P 190W | Ningbo Solar Electric Power TPB156x156-54-P 195W | Ningbo Solar Electric Power TPB125x125-96-P 200W | Ningbo Solar Electric Power TPB156x156-54-P 200W | Ningbo Solar Electric Power TPB156x156-60-P 200W | Ningbo Solar Electric Power TPB156x156-60-P 205W | Ningbo Solar Electric Power TPB125x125-96-P 210W | Ningbo Solar Electric Power TPB156x156-60-P 210W | Ningbo Solar Electric Power TPB156x156-60-P 215W | Ningbo Solar Electric Power TPB125x125-96-P 220W | Ningbo Solar Electric Power TPB156x156-60-P 220W | Ningbo Solar Electric Power TPB156x156-60-P 225W | Ningbo Solar Electric Power TPB125x125-96-P 230W | Ningbo Solar Electric Power TPB156x156-60-P 230W | Ningbo Solar Electric Power TPB156x156-72-P 230W | Ningbo Solar Electric Power TPB125x125-96-P 240W | Ningbo Solar Electric Power TPB156x156-72-P 240W | Ningbo Solar Electric Power TPB156x156-72-P 250W | Ningbo Solar Electric Power TPB156x156-72-P 255W | Ningbo Solar Electric Power TPB156x156-72-P 260W | Ningbo Solar Electric Power TPB156x156-72-P 270W | Ningbo Solar Electric Power TPB156x156-72-P 280W | Ningbo Ulica Solar Science & Technology 165(35) D UL811x1581 | Ningbo Ulica Solar Science & Technology UL-180D | Ningbo Ulica Solar Science & Technology UL-185D | Ningbo Ulica Solar Science & Technology UL-190D | Ningbo Ulica Solar Science & Technology 230(35) D UL997x1953 | Ningbo Ulica Solar Science & Technology UL-230D | Ningbo Ulica Solar Science & Technology UL-230P | Ningbo Ulica Solar Science & Technology UL-235D | Ningbo Ulica Solar Science & Technology UL-235P | Ningbo Ulica Solar Science & Technology UL-240D | Ningbo Ulica Solar Science & Technology UL-240D-96 | Ningbo Ulica Solar Science & Technology UL-240P | Ningbo Ulica Solar Science & Technology UL-245D | Ningbo Ulica Solar Science & Technology UL-245D-96 | Ningbo Ulica Solar Science & Technology UL-245P | Ningbo Ulica Solar Science & Technology UL-250D | Ningbo Ulica Solar Science & Technology UL-250D-96 | Ningbo Ulica Solar Science & Technology UL-250P | Ningbo Ulica Solar Science & Technology UL-255D-96 | Ningbo Ulica Solar Science & Technology UL-260D-96 | Ningbo Ulica Solar Science & Technology UL-275D | Ningbo Ulica Solar Science & Technology UL-275P | Ningbo Ulica Solar Science & Technology UL-280D | Ningbo Ulica Solar Science & Technology UL-280P | Ningbo Ulica Solar Science & Technology UL-285D | Ningbo Ulica Solar Science & Technology UL-285P | Ningbo Ulica Solar Science & Technology UL-290D | Ningbo Ulica Solar Science & Technology UL-290P | Ningbo Ulica Solar Science & Technology UL-295D | Ningbo Ulica Solar Science & Technology UL-295P | Ningbo Ulica Solar Science & Technology UL-300D | Ningxia Yinxing Energy Photovoltaic Equipment Manufact YXGF-180M72 | Ningxia Yinxing Energy Photovoltaic Equipment Manufact YXGF-185M72 | Ningxia Yinxing Energy Photovoltaic Equipment Manufact YXGF-190M72 | Ningxia Yinxing Energy Photovoltaic Equipment Manufact YXGF-195M72 | Ningxia Yinxing Energy Photovoltaic Equipment Manufact YXGF-200M72 | Ningxia Yinxing Energy Photovoltaic Equipment Manufact YXGF-205M72 | Ningxia Yinxing Energy Photovoltaic Equipment Manufact YXGF-210M72 | Ningxia Yinxing Energy Photovoltaic Equipment Manufact YXGF-230P60 | Ningxia Yinxing Energy Photovoltaic Equipment Manufact YXGF-235P60 | Ningxia Yinxing Energy Photovoltaic Equipment Manufact YXGF-240P60 | Ningxia Yinxing Energy Photovoltaic Equipment Manufact YXGF-245P60 | Ningxia Yinxing Energy Photovoltaic Equipment Manufact YXGF-250P60 | Ningxia Yinxing Energy Photovoltaic Equipment Manufact YXGF-255P60 | Ningxia Yinxing Energy Photovoltaic Equipment Manufact YXGF-275P72 | Ningxia Yinxing Energy Photovoltaic Equipment Manufact YXGF-280P72 | Ningxia Yinxing Energy Photovoltaic Equipment Manufact YXGF-285P72 | Ningxia Yinxing Energy Photovoltaic Equipment Manufact YXGF-290M72 | Ningxia Yinxing Energy Photovoltaic Equipment Manufact YXGF-290P72 | Ningxia Yinxing Energy Photovoltaic Equipment Manufact YXGF-295M72 | Ningxia Yinxing Energy Photovoltaic Equipment Manufact YXGF-295P72 | Ningxia Yinxing Energy Photovoltaic Equipment Manufact YXGF-300M72 | Ningxia Yinxing Energy Photovoltaic Equipment Manufact YXGF-300P72 | Ningxia Yinxing Energy Photovoltaic Equipment Manufact YXGF-305M72 | Ningxia Yinxing Energy Photovoltaic Equipment Manufact YXGF-305P72 | Nu-Cell Technologies NCT250-5M812 | Nu-Cell Technologies NCT255-5M812 | Nu-Cell Technologies NCT260-5M812 | Nu-Cell Technologies NCT265-5M812 | Nu-Cell Technologies NCT270-5M812 | Nu-Cell Technologies NCT270-6M612 | Nu-Cell Technologies NCT275-6M612 | Nu-Cell Technologies NCT280-6M612 | Nu-Cell Technologies NCT285-6M612 | Nu-Cell Technologies NCT290-6M612 | Nusun Solar NS280-6M7 | Panasonic Eco Solutions Canada PE240M-BBB | Panasonic Eco Solutions Canada PE240P-BBB | Panasonic Eco Solutions Canada PE245M-BBB | Panasonic Eco Solutions Canada PE245P-BBB | Panasonic Eco Solutions Canada PE250M-BBB | Panasonic Eco Solutions Canada PE250P-BBB | Panasonic Eco Solutions Canada PE255M-BBB | Panasonic Eco Solutions Canada PE255P-BBB | Panasonic Eco Solutions Canada PE260M-BBB | Panasonic Eco Solutions Canada PE290M-BBB | Panasonic Eco Solutions Canada PE290P-BBB | Panasonic Eco Solutions Canada PE295M-BBB | Panasonic Eco Solutions Canada PE295P-BBB | Panasonic Eco Solutions Canada PE300M-BBB | Panasonic Eco Solutions Canada PE300P-BBB | Panasonic Eco Solutions Canada PE305M-BBB | Panasonic Eco Solutions Canada PE305P-BBB | Panasonic Eco Solutions Canada PE310M-BBB | Panasonic Eco Solutions Canada PE310P-BBB | Panasonic Eco Solutions Canada PE315M-BBB | Panasonic Eco Solutions Canada PE320M-BBB | Perfect Source Technology PST 170 3GP48 | Perfect Source Technology PST 176 3GP48 | Perfect Source Technology PST 182 3GM48 | Perfect Source Technology PST 182 3GP48 | Perfect Source Technology PST 188 3GM48 | Perfect Source Technology PST 188 3GP48 | Perfect Source Technology PST 194 3GM48 | Perfect Source Technology PST 194 3GP48 | Perfect Source Technology PST 194 3GP54 | Perfect Source Technology PST 200 3GM48 | Perfect Source Technology PST 200 3GP48 | Perfect Source Technology PST 200 3GP54 | Perfect Source Technology PST 206 3GM48 | Perfect Source Technology PST 206 3GM54 | Perfect Source Technology PST 206 3GP54 | Perfect Source Technology PST 212 3GM48 | Perfect Source Technology PST 212 3GM54 | Perfect Source Technology PST 212 3GP54 | Perfect Source Technology PST 212GT | Perfect Source Technology PST 218 3GM54 | Perfect Source Technology PST 218 3GP54 | Perfect Source Technology PST 218 3GP60 | Perfect Source Technology PST 218GT | Perfect Source Technology PST 224 3GM54 | Perfect Source Technology PST 224 3GM60 | Perfect Source Technology PST 224 3GP60 | Perfect Source Technology PST 224GT | Perfect Source Technology PST 230 3GM54 | Perfect Source Technology PST 230 3GM60 | Perfect Source Technology PST 230 3GP60 | Perfect Source Technology PST 230GT | Perfect Source Technology PST 236 3GM54 | Perfect Source Technology PST 236 3GM60 | Perfect Source Technology PST 236 3GP60 | Perfect Source Technology PST 236GT | Perfect Source Technology PST 242 3GM60 | Perfect Source Technology PST 242 3GP60 | Perfect Source Technology PST 248 3GM60 | Perfect Source Technology PST 248 3GP60 | Perfect Source Technology PST 254 3GM60 | Perfect Source Technology PST 254 3GP60 | Perfectenergy (Shanghai) PEM-160-180-72M | Perlight Solar PLM-175M-72 | Perlight Solar PLM-185M-72 | Perlight Solar PLM-205P-60 | Perlight Solar PLM-210P-60 | Perlight Solar PLM-215P-60 | Perlight Solar PLM-215P-60US1 | Perlight Solar PLM-220P-60 | Perlight Solar PLM-220P-60US1 | Perlight Solar PLM-225P-60 | Perlight Solar PLM-225P-60US1 | Perlight Solar PLM-230P-60 | Perlight Solar PLM-230P-60US1 | Perlight Solar PLM-235M-60US1 | Perlight Solar PLM-235P-60 | Perlight Solar PLM-240M-60 | Perlight Solar PLM-240M-60US1 | Perlight Solar PLM-240P-60 | Perlight Solar PLM-245M-60 | Perlight Solar PLM-245M-60US1 | Perlight Solar PLM-250M-60 | Perlight Solar PLM-250M-60US1 | Perlight Solar PLM-255M-60 | Perlight Solar PLM-270P-72 | Perlight Solar PLM-275P-72 | Perlight Solar PLM-280P-72 | Perlight Solar PLM-285P-72 | Perlight Solar PLM-290M-72 | Perlight Solar PLM-290P-72 | Perlight Solar PLM-295M-72 | Perlight Solar PLM-300M-72 | Perlight Solar PLM-305M-72 | Perlight Solar PLM-335M-80US1 | Perlight Solar PLM-340M-80US1 | Perlight Solar PLM-345M-80US1 | Perlight Solar PLM-350M-80US1 | Pevafersa America IP-220 GG | Pevafersa America IP-225 GG | Pevafersa America IP-230 GG | Pevafersa America IP-235 GG | Philadelphia Solar PS-M36S-90 | Philadelphia Solar PS-M36S-95 | Philadelphia Solar PS-P36-130 | Philadelphia Solar PS-P36-135 | Philadelphia Solar PS-P36-140 | Philadelphia Solar PS-P36-145 | Philadelphia Solar PS-M72S-180 | Philadelphia Solar PS-M72S-185 | Philadelphia Solar PS-M72S-190 | Philadelphia Solar PS-P54-205 | Philadelphia Solar PS-P54-210 | Philadelphia Solar PS-P54-215 | Philadelphia Solar PS-P54-220 | Philadelphia Solar PS-P60-220 | Philadelphia Solar PS-P54-225 | Philadelphia Solar PS-P60-230 | Philadelphia Solar PS-P60-235 | Philadelphia Solar PS-P60-240 | Philadelphia Solar PS-P60-245 | Philadelphia Solar PS-P60-250 | Philadelphia Solar PS-P72-270 | Philadelphia Solar PS-P72-275 | Philadelphia Solar PS-P72-280 | Philadelphia Solar PS-P72-285 | Philadelphia Solar PS-P72-290 | Phono Solar Technology PS160M-24-F | Phono Solar Technology PS165M-24-F | Phono Solar Technology PS170M-24-F | Phono Solar Technology PS180M-24-F | Phono Solar Technology PS185M-24-F | Phono Solar Technology PS190M-24-F | Phono Solar Technology PS195M-24-F | Phono Solar Technology PS200M-24-F | Phono Solar Technology PS210M-20-U | Phono Solar Technology PS210P-20-U | Phono Solar Technology PS215M-20-U | Phono Solar Technology PS215P-20-U | Phono Solar Technology PS220M-20-U | Phono Solar Technology PS220P-20-U | Phono Solar Technology PS225M-20-U | Phono Solar Technology PS225P-20-U | Phono Solar Technology PS230M-20-U | Phono Solar Technology PS230MB-20-U | Phono Solar Technology PS230P-20-U | Phono Solar Technology PS230PB-20-U | Phono Solar Technology PS235M-20-U | Phono Solar Technology PS235MB-20-U | Phono Solar Technology PS235P-20-U | Phono Solar Technology PS235PB-20-U | Phono Solar Technology PS240M-20-U | Phono Solar Technology PS240M-20-U-AC | Phono Solar Technology PS240MB-20-U | Phono Solar Technology PS240P-20-U | Phono Solar Technology PS240P-20-U-AC | Phono Solar Technology PS240PB-20-U | Phono Solar Technology PS245M | Phono Solar Technology PS245M-20-U | Phono Solar Technology PS245M-20-U-AC | Phono Solar Technology PS245MB-20-U | Phono Solar Technology PS245P-20-U | Phono Solar Technology PS245P-20-U-AC | Phono Solar Technology PS245PB-20-U | Phono Solar Technology PS250M | Phono Solar Technology PS250M-20-U | Phono Solar Technology PS250M-20-U-AC | Phono Solar Technology PS250MB-20-U | Phono Solar Technology PS250P-20-U | Phono Solar Technology PS250P-20-U-AC | Phono Solar Technology PS250PB-20-U | Phono Solar Technology PS255M-20-U | Phono Solar Technology PS255M-20-U-AC | Phono Solar Technology PS255MB-20-U | Phono Solar Technology PS255P-20-U | Phono Solar Technology PS255P-20-U-AC | Phono Solar Technology PS255PB-20-U | Phono Solar Technology PS260M-20-U | Phono Solar Technology PS260M-20-U-AC | Phono Solar Technology PS260M-24-T | Phono Solar Technology PS260MB-20-U | Phono Solar Technology PS260P-20-U | Phono Solar Technology PS260P-20-U-AC | Phono Solar Technology PS260P-24-T | Phono Solar Technology PS260PB-20-U | Phono Solar Technology PS270M-24-T | Phono Solar Technology PS270P-24-T | Phono Solar Technology PS280M-24-T | Phono Solar Technology PS280MB-24-T | Phono Solar Technology PS280P-24-T | Phono Solar Technology PS280PB-24-T | Phono Solar Technology PS285M-24-T | Phono Solar Technology PS285MB-24-T | Phono Solar Technology PS285P-24-T | Phono Solar Technology PS285PB-24-T | Phono Solar Technology PS290M-24-T | Phono Solar Technology PS290MB-24-T | Phono Solar Technology PS290P-24-T | Phono Solar Technology PS290PB-24-T | Phono Solar Technology PS295M-24-T | Phono Solar Technology PS295MB-24-T | Phono Solar Technology PS295P-24-T | Phono Solar Technology PS295PB-24-T | Phono Solar Technology PS300M-24-T | Phono Solar Technology PS300MB-24-T | Phono Solar Technology PS300P-24-T | Phono Solar Technology PS300PB-24-T | Phono Solar Technology PS305M-24-T | Phono Solar Technology PS305MB-24-T | Phono Solar Technology PS305P-24-T | Phono Solar Technology PS305PB-24-T | Phono Solar Technology PS310M-24-T | Phono Solar Technology PS310MB-24-T | Phono Solar Technology PS310P-24-T | Phono Solar Technology PS310PB-24-T | Phono Solar Technology PS315M-24-T | Phono Solar Technology PS315MB-24-T | Phono Solar Technology PS315P-24-T | Phono Solar Technology PS315PB-24-T | Phono Solar Technology PS320MB-24-T | Phono Solar Technology PS320PB-24-T | Photowatt Ontario PW2300-220 | Photowatt Ontario PW2300-225 | Photowatt Ontario PW2300-230 | Photowatt Ontario PW2300-235 | Photowatt Ontario PW2300-240 | Photowatt Ontario PW2300-245 | Photowatt Ontario PW2300-250 | Photowatt Ontario PW2300-255 | Photowatt Ontario PW2750-265 | Photowatt Ontario PW2750-270 | Photowatt Ontario PW2750-275 | Photowatt Ontario PW2750-280 | Photowatt Ontario PW2750-285 | Polar Photovoltaics TFSM-T-0 | Polar Photovoltaics TFSM-T-0X | Polar Photovoltaics TFSM-T-1 | Polar Photovoltaics TFSM-T-1X | Polar Photovoltaics TFSM-T-2 | Polar Photovoltaics TFSM-T-2X | Polar Photovoltaics TFSM-T-3 | Polar Photovoltaics TFSM-T-3X | Polar Photovoltaics TFSM-T-4 | Polar Photovoltaics TFSM-T-4X | Polar Photovoltaics TFSM-T-5 | Polar Photovoltaics TFSM-T-5X | Powercom PPV-115M6 | Powercom PPV-115S6 | Powercom PPV-120M6 | Powercom PPV-120S6 | Powercom PPV-125M6 | Powercom PPV-125S6 | Powercom PPV-130M6L | Powercom PPV-140M6 | Powercom PPV-145M6 | Powercom PPV-145S6 | Powercom PPV-150M6 | Powercom PPV-150S6 | Powercom PPV-155M6 | Powercom PPV-155S6 | Powercom PPV-175M6 | Powercom PPV-180M6L | Powercom PPV-180M6 | Powercom PPV-180S6 | Powercom PPV-185M6 | Powercom PPV-185S6 | Powercom PPV-190M6 | Powercom PPV-190S6 | Powercom PPV-195M6 | Powercom PPV-200M6 | Powercom PPV-205M6 | Powercom PPV-210M6 | Powercom PPV-210M6L | Powercom PPV-215M6 | Powercom PPV-220M6 | Powercom PPV-220M6L | Powercom PPV-230M6L | Powercom PPV-225M6 | Powercom PPV-225S6 | Powercom PPV-230M6 | Powercom PPV-230S6 | Powercom PPV-235M6 | Powercom PPV-235S6 | Powercom PPV-240M6 | Powercom PPV-260M6 | Powercom PPV-260S6 | Powercom PPV-265M6 | Powercom PPV-265S6 | Powercom PPV-270M6 | Powercom PPV-270S6 | Powercom PPV-275M6 | Powercom PPV-275S6 | Powercom PPV-285S6 | Powercom PPV-290S6 | Prism Solar Technologies B 150 | Prism Solar Technologies HB 180 | Prism Solar Technologies B 245 | Pythagoras Solar Midi PVGU Window | Pythagoras Solar Large PVGU Window | Quantum Technologies QS 215W-60-156 AP 2BB | Quantum Technologies QS 220W-60-156 AP 2BB | Quantum Technologies QS 220W-60-156 SP 2BB | Quantum Technologies QS 225W-60-156 AP 2BB | Quantum Technologies QS 225W-60-156 SP 2BB | Quantum Technologies QS 225W-60-256 EM 3BB | Quantum Technologies QS 230W-60-156 SP 2BB | Realforce Power RF-215P60 | Realforce Power RF-220P60 | Realforce Power RF-225P60 | Realforce Power RF-230P60 | Realforce Power RF-235P60 | Realforce Power RF-240P60 | Realforce Power RF-245P60 | Realforce Power RF-250P60 | Realforce Power RF-255P72 | Realforce Power RF-260P72 | Realforce Power RF-265P72 | Realforce Power RF-270P72 | Realforce Power RF-275P72 | Realforce Power RF-280P72 | Realforce Power RF-285P72 | Realforce Power RF-290P72 | Realforce Power RF-295P72 | REC ScanModule SCM205 | REC ScanModule SCM210 | REC ScanModule SCM215 | REC ScanModule SCM220 | REC ScanModule SCM225 | REC Solar REC205AE-US | REC Solar REC205AE-US (BLK) | REC Solar REC205PE | REC Solar REC205PE (BLK) | REC Solar REC205PE Q2 | REC Solar REC205PE Q3 | REC Solar REC205PE-US | REC Solar REC205PE-US (BLK) | REC Solar REC210AE-US | REC Solar REC210AE-US (BLK) | REC Solar REC210PE | REC Solar REC210PE (BLK) | REC Solar REC210PE Q2 | REC Solar REC210PE Q3 | REC Solar REC210PE-US | REC Solar REC210PE-US (BLK) | REC Solar REC215AE-US | REC Solar REC215AE-US (BLK) | REC Solar REC215PE | REC Solar REC215PE (BLK) | REC Solar REC215PE-US | REC Solar REC215PE-US (BLK) | REC Solar REC220AE-US | REC Solar REC220AE-US (BLK) | REC Solar REC220PE | REC Solar REC220PE (BLK) | REC Solar REC220PE-US | REC Solar REC220PE-US (BLK) | REC Solar REC225AE-US | REC Solar REC225AE-US (BLK) | REC Solar REC225PE | REC Solar REC225PE (BLK) | REC Solar REC225PE-US | REC Solar REC225PE-US (BLK) | REC Solar REC230AE-US | REC Solar REC230AE-US (BLK) | REC Solar REC230PE | REC Solar REC230PE (BLK) | REC Solar REC230PE-US | REC Solar REC230PE-US (BLK) | REC Solar REC235PE | REC Solar REC235PE (BLK) | REC Solar REC235PE ECO | REC Solar REC235PE Q2 | REC Solar REC235PE Q2 ECO | REC Solar REC235PE Q3 | REC Solar REC235PE Q3 ECO | REC Solar REC235PE(BLK) ECO | REC Solar REC235PE-US | REC Solar REC235PE-US (BLK) | REC Solar REC235PE-US ECO | REC Solar REC235PE-US(BLK) ECO | REC Solar REC240PE | REC Solar REC240PE (BLK) | REC Solar REC240PE ECO | REC Solar REC240PE Q2 | REC Solar REC240PE Q2 ECO | REC Solar REC240PE Q3 | REC Solar REC240PE Q3 ECO | REC Solar REC240PE(BLK) ECO | REC Solar REC240PE-US | REC Solar REC240PE-US (BLK) | REC Solar REC240PE-US ECO | REC Solar REC240PE-US(BLK) ECO | REC Solar REC245PE | REC Solar REC245PE (BLK) | REC Solar REC245PE ECO | REC Solar REC245PE Q2 | REC Solar REC245PE Q2 ECO | REC Solar REC245PE Q3 | REC Solar REC245PE Q3 ECO | REC Solar REC245PE(BLK) ECO | REC Solar REC245PE-US | REC Solar REC245PE-US (BLK) | REC Solar REC245PE-US ECO | REC Solar REC245PE-US(BLK) ECO | REC Solar REC250PE | REC Solar REC250PE (BLK) | REC Solar REC250PE ECO | REC Solar REC250PE Q2 | REC Solar REC250PE Q2 ECO | REC Solar REC250PE Q3 | REC Solar REC250PE Q3 ECO | REC Solar REC250PE(BLK) ECO | REC Solar REC250PE-US | REC Solar REC250PE-US (BLK) | REC Solar REC250PE-US ECO | REC Solar REC250PE-US(BLK) ECO | REC Solar REC255PE | REC Solar REC255PE Q2 | REC Solar REC255PE Q3 | REC Solar REC255PE(BLK) | REC Solar REC255PE-US | REC Solar REC255PE-US(BLK) | REC Solar REC260PE | REC Solar REC260PE Q2 | REC Solar REC260PE Q3 | REC Solar REC260PE(BLK) | REC Solar REC260PE-US | REC Solar REC260PE-US(BLK) | Renesola America JC180S-24-Db | Renesola America JC185S-24-Db | Renesola America JC190S-24-Db | Renesola America JC195S-24-Db | Renesola America JC200S-24-Db | Renesola America JC220M-24-Bb | Renesola America JC225M-24-Bb | Renesola America JC225S-24-Bb | Renesola America JC230M-24-Bb | Renesola America JC230S-24-Bb | Renesola America JC235M-24-Bb | Renesola America JC235S-24-Bb | Renesola America JC240M-24-Bb | Renesola America JC240M-24-Bb-b | Renesola America JC240S-24-Bb | Renesola America JC240S-24-Bb-b | Renesola America JC245M-24-Bb | Renesola America JC245M-24-Bb-b | Renesola America JC245S-24-Bb | Renesola America JC245S-24-Bb-b | Renesola America JC250M-24-Bb | Renesola America JC250M-24-Bb-b | Renesola America JC250S-24-Bb | Renesola America JC250S-24-Bb-b | Renesola America JC255M-24-Bb | Renesola America JC255M-24-Bb-b | Renesola America JC255S-24-Bb | Renesola America JC255S-24-Bb-b | Renesola America JC260S-24-Bb | Renesola America JC260S-24-Bb-b | Renesola America JC265S-24-Ab | Renesola America JC270M-24-Ab | Renesola America JC270S-24-Ab | Renesola America JC275M-24-Ab | Renesola America JC275S-24-Ab | Renesola America JC280M-24-Ab | Renesola America JC280S-24-Ab | Renesola America JC285M-24-Ab | Renesola America JC285M-24-Ab-b | Renesola America JC285S-24-Ab | Renesola America JC290M-24-Ab | Renesola America JC290M-24-Ab-b | Renesola America JC290S-24-Ab | Renesola America JC295M-24-Ab | Renesola America JC295M-24-Ab-b | Renesola America JC295S-24-Ab | Renesola America JC300M-24-Ab | Renesola America JC300M-24-Ab-b | Renesola America JC300S-24-Ab | Renesola America JC305M-24-Ab | Renesola America JC305M-24-Ab-b | Renesola Jiangsu JC180S-24-Db | Renesola Jiangsu JC185S-24-Db | Renesola Jiangsu JC190S-24-Db | Renesola Jiangsu JC195S-24-Db | Renesola Jiangsu JC200S-24-Db | Renesola Jiangsu JC220M-24-Bx | Renesola Jiangsu JC225M-24-Bx | Renesola Jiangsu JC225S-24-Bb | Renesola Jiangsu JC230M-24-Bb | Renesola Jiangsu JC230S-24-Bb | Renesola Jiangsu JC235M-24-Bx | Renesola Jiangsu JC235S-24-Bb | Renesola Jiangsu JC240M-24-Bx | Renesola Jiangsu JC240M-24-Bx-b | Renesola Jiangsu JC240M-24-Bxh | Renesola Jiangsu JC240M-24-Bxh-b | Renesola Jiangsu JC240S-24-Bb | ReneSola Jiangsu JC240S-24-Bb-b | ReneSola Jiangsu JC245M-24-Bbv | Renesola Jiangsu JC245M-24-Bx | Renesola Jiangsu JC245M-24-Bx-b | Renesola Jiangsu JC245M-24-Bxh | Renesola Jiangsu JC245M-24-Bxh-b | Renesola Jiangsu JC245S-24-Bb | ReneSola Jiangsu JC245S-24-Bb-b | Renesola Jiangsu JC245S-24-Bbh | Renesola Jiangsu JC245S-24-Bbh-b | ReneSola Jiangsu JC250M-24-Bbv | Renesola Jiangsu JC250M-24-Bx | Renesola Jiangsu JC250M-24-Bx-b | Renesola Jiangsu JC250M-24-Bxh | Renesola Jiangsu JC250M-24-Bxh-b | Renesola Jiangsu JC250S-24-Bb | ReneSola Jiangsu JC250S-24-Bb-b | Renesola Jiangsu JC250S-24-Bbh | Renesola Jiangsu JC250S-24-Bbh-b | ReneSola Jiangsu JC255M-24-Bbv | Renesola Jiangsu JC255M-24-Bx | Renesola Jiangsu JC255M-24-Bx-b | Renesola Jiangsu JC255M-24-Bxh | Renesola Jiangsu JC255M-24-Bxh-b | Renesola Jiangsu JC255S-24-Bb | ReneSola Jiangsu JC255S-24-Bb-b | Renesola Jiangsu JC255S-24-Bbh | Renesola Jiangsu JC255S-24-Bbh-b | ReneSola Jiangsu JC260M-24-Bbv | Renesola Jiangsu JC260M-24-Bx | Renesola Jiangsu JC260M-24-Bx-b | Renesola Jiangsu JC260M-24-Bxh | Renesola Jiangsu JC260M-24-Bxh-b | Renesola Jiangsu JC260S-24-Bb | ReneSola Jiangsu JC260S-24-Bb-b | ReneSola Jiangsu JC265M-24-Bbv | Renesola Jiangsu JC265S-24-Ab | Renesola Jiangsu JC270M-24-Ax | Renesola Jiangsu JC270S-24-Ab | Renesola Jiangsu JC275M-24-Ax | Renesola Jiangsu JC275S-24-Ab | Renesola Jiangsu JC280M-24-Ax | Renesola Jiangsu JC280S-24-Ab | ReneSola Jiangsu JC285M-24-Abv | Renesola Jiangsu JC285M-24-Ax | Renesola Jiangsu JC285M-24-Ax-b | Renesola Jiangsu JC285M-24-Axh | Renesola Jiangsu JC285M-24-Axh-b | Renesola Jiangsu JC285S-24-Ab | ReneSola Jiangsu JC290M-24-Abv | Renesola Jiangsu JC290M-24-Ax | Renesola Jiangsu JC290M-24-Ax-b | Renesola Jiangsu JC290M-24-Axh | Renesola Jiangsu JC290M-24-Axh-b | Renesola Jiangsu JC290S-24-Ab | Renesola Jiangsu JC290S-24-Abh | Renesola Jiangsu JC290S-24-Abh-b | ReneSola Jiangsu JC295M-24-Abv | Renesola Jiangsu JC295M-24-Ax | Renesola Jiangsu JC295M-24-Ax-b | Renesola Jiangsu JC295M-24-Axh | Renesola Jiangsu JC295M-24-Axh-b | Renesola Jiangsu JC295S-24-Ab | Renesola Jiangsu JC295S-24-Abh | Renesola Jiangsu JC295S-24-Abh-b | ReneSola Jiangsu JC300M-24-Abv | Renesola Jiangsu JC300M-24-Ax | Renesola Jiangsu JC300M-24-Ax-b | Renesola Jiangsu JC300M-24-Axh | Renesola Jiangsu JC300M-24-Axh-b | Renesola Jiangsu JC300S-24-Ab | Renesola Jiangsu JC300S-24-Abh | Renesola Jiangsu JC300S-24-Abh-b | ReneSola Jiangsu JC305M-24-Abv | Renesola Jiangsu JC305M-24-Ax | Renesola Jiangsu JC305M-24-Ax-b | Renesola Jiangsu JC305M-24-Axh | Renesola Jiangsu JC305M-24-Axh-b | Renesola Jiangsu JC305S-24-Ab | Renesola Jiangsu JC305S-24-Abh | Renesola Jiangsu JC305S-24-Abh-b | ReneSola Jiangsu JC310M-24-Abv | Renesola Jiangsu JC310M-24-Ax-b | Renesola Jiangsu JC310M-24-Axh | Renesola Jiangsu JC310M-24-Axh-b | Renesola Jiangsu JC310S-24-Abh | Renesola Jiangsu JC310S-24-Abh-b | ReneSola Jiangsu JC315M-24-Abv | Renesola Jiangsu JC315M-24-Ax-b | Renesola Jiangsu JC315M-24-Axh | Renesola Jiangsu JC315M-24-Axh-b | Renesola Jiangsu JC315S-24-Abh | Renesola Jiangsu JC315S-24-Abh-b | Renesola Jiangsu JC320S-24-Abh | Renesola Jiangsu JC320S-24-Abh-b | Renogy RNG-175D | Renogy RNG-180D | Renogy RNG-185D | Renogy RNG-215P | Renogy RNG-220P | Renogy RNG-225D | Renogy RNG-225P | Renogy RNG-230D | Renogy RNG-230P | Renogy RNG-235D | Renogy RNG-235P | Renogy RNG-240D | Renogy RNG-245D | Renogy RNG-250P | Renogy RNG-260D | Renogy RNG-260P | Renogy RNG-265D | Renogy RNG-270D | Renogy RNG-270P | Renogy RNG-275D | Renogy RNG-280D | Renogy RNG-285D | Renogy RNG-290D | Resonix EPML120W6H | Resonix EPMN120W6H | Resonix EPML130W6H | Resonix EPMN130W6H | Resonix EPML150W6H | Resonix EPMN150W6H | Resonix EPML180W6H | Resonix EPMN180W6H | Resonix EPML185W6H | Resonix EPMN185W6H | Resonix EPML220W6H | Resonix EPML225W6H | Resonix EPMN225W6H | Resonix EPML275W6H | Resonix EPMN275W6H | Risen Energy SYP-85S | Risen Energy SYP-110S | Risen Energy SYP-160S | Risen Energy SYP-165S | Risen Energy SYP-170S | Risen Energy SYP-175S | Risen Energy SYP-180S | Risen Energy SYP-185S | Risen Energy SYP-190S | Risen Energy SYP-195S | Risen Energy SYP200P | Risen Energy SYP-200S | Risen Energy SYP-200W | Risen Energy SYP210M | Risen Energy SYP210P | Risen Energy SYP-210S | Risen Energy SYP220M | Risen Energy SYP220P | Risen Energy SYP230M | Risen Energy SYP230P | Risen Energy SYP240M | Risen Energy SYP240P | Risen Energy SYP250M | Risen Energy SYP250P | Risen Energy SYP260M | Risen Energy SYP260P | Risen Energy SYP270M | Risen Energy SYP270P | Risen Energy SYP280M | Risen Energy SYP280P | Risen Energy SYP290M | Risen Energy SYP300M | Risen Energy SYP305M | Ritek PM130 | Ritek MM135 | Ritek PM135 | Ritek MM140 | Ritek PM140 | Ritek MM145 | Ritek PM175 | Ritek MM180 | Ritek PM180 | Ritek MM185 | Ritek PM185 | Ritek MM190 | Ritek PM190 | Ritek MM195 | Ritek PM195 | Ritek MM200 | Ritek PM200 | Ritek MM205 | Ritek PM205 | Ritek MM210 | Ritek PM210 | Ritek MM215 | Ritek PM215 | Ritek MM220 | Ritek PM220 | Ritek MM225 | Ritek PM225 | Ritek MM230 | Ritek PM230 | Ritek MM235 | Ritek PM235 | Ritek MM240 | Ritek PM240 | Ritek PM270T | Ritek PM275 | Ritek PM275T | Ritek PM280 | Ritek PM280T | Ritek MM285T | Ritek PM285 | Ritek PM285T | Ritek MM290T | Ritek PM290 | Ritek PM290T | Ritek MM295T | Ritek PM295 | Ritek MM300T | Ritek MM305T | Saint Gobain Solar SKA180M72-WN | Saint Gobain Solar SKA185M72-WN | Saint Gobain Solar SKA190M72-WN | Saint Gobain Solar SKA220P60-WN | Saint Gobain Solar SKA225M60-WN | Saint Gobain Solar SKA225P60-WN | Saint Gobain Solar SKA230M60-WN | Saint Gobain Solar SKA230P60-WN | Saint Gobain Solar SKA235P60-WN | Saint Gobain Solar SKA240M60-WN | Saint Gobain Solar SKA240P60-WN | Saint Gobain Solar SKA245M60-WN | Saint Gobain Solar SKA250M60-WN | Samsung SDI LPC235SM-02 | Samsung SDI LPC235SM-08 | Samsung SDI LPC238SM-02 | Samsung SDI LPC238SM-08 | Samsung SDI LPC241SM-02 | Samsung SDI LPC241SM-08 | Samsung SDI LPC244SM-02 | Samsung SDI LPC244SM-08 | Samsung SDI PV-MBA1BG244 | Samsung SDI PV-MBA1CG244 | Samsung SDI LPC247SM-08 | Samsung SDI PV-MBA1BG247 | Samsung SDI PV-MBA1CG247 | Samsung SDI LPC250SM-08 | Samsung SDI PV-MBA1BG250 | Samsung SDI PV-MBA1CG250 | Samsung SDI PV-MBA1BG255 | Samsung SDI PV-MBA1CG255 | Sanyo Electric of Panasonic Group HIP-186DA3 | Sanyo Electric of Panasonic Group VBHB186DA03 | Sanyo Electric of Panasonic Group VBHB186DA03B | Sanyo Electric of Panasonic Group HIP-190DA3 | Sanyo Electric of Panasonic Group VBHB190DA03 | Sanyo Electric of Panasonic Group VBHB190DA03B | Sanyo Electric of Panasonic Group HIP-195BA20 | Sanyo Electric of Panasonic Group HIP-195DA3 | Sanyo Electric of Panasonic Group VBHB195AA20 | Sanyo Electric of Panasonic Group VBHB195AA20B | Sanyo Electric of Panasonic Group VBHB195DA03 | Sanyo Electric of Panasonic Group VBHB195DA03B | Sanyo Electric of Panasonic Group HIP-200BA20 | Sanyo Electric of Panasonic Group VBHB200AA20 | Sanyo Electric of Panasonic Group VBHB200AA20B | Sanyo Electric of Panasonic Group HIT-N210A01 | Sanyo Electric of Panasonic Group VBHN210AA01 | Sanyo Electric of Panasonic Group VBHN210AA01B | Sanyo Electric of Panasonic Group HIP-215NKHA6 | Sanyo Electric of Panasonic Group HIT-N215A01 | Sanyo Electric of Panasonic Group VBHN215AA01 | Sanyo Electric of Panasonic Group VBHN215AA01B | Sanyo Electric of Panasonic Group VBHN215AA06 | Sanyo Electric of Panasonic Group VBHN215AA06B | Sanyo Electric of Panasonic Group HIT-N220A01 | Sanyo Electric of Panasonic Group VBHN220AA01 | Sanyo Electric of Panasonic Group VBHN220AA01B | Sanyo Electric of Panasonic Group VBHN220SA06 | Sanyo Electric of Panasonic Group VBHN220SA06B | Sanyo Electric of Panasonic Group HIT-N225A01 | Sanyo Electric of Panasonic Group VBHN225AA01 | Sanyo Electric of Panasonic Group VBHN225AA01B | Sanyo Electric of Panasonic Group VBHN225SA06 | Sanyo Electric of Panasonic Group VBHN225SA06B | Sanyo Electric of Panasonic Group VBHN230SA04 | Sanyo Electric of Panasonic Group VBHN230SA04B | Sanyo Electric of Panasonic Group VBHN230SA06 | Sanyo Electric of Panasonic Group VBHN230SA06B | Sanyo Electric of Panasonic Group VBHN230SA11 | Sanyo Electric of Panasonic Group VBHN230SA11B | Sanyo Electric of Panasonic Group VBHN235SA04 | Sanyo Electric of Panasonic Group VBHN235SA04B | Sanyo Electric of Panasonic Group VBHN235SA06 | Sanyo Electric of Panasonic Group VBHN235SA06B | Sanyo Electric of Panasonic Group VBHN235SA11 | Sanyo Electric of Panasonic Group VBHN235SA11B | Sanyo Electric of Panasonic Group VBHN240SA04 | Sanyo Electric of Panasonic Group VBHN240SA04B | Sanyo Electric of Panasonic Group VBHN240SA06 | Sanyo Electric of Panasonic Group VBHN240SA06B | Sanyo Electric of Panasonic Group VBHN240SA11 | Sanyo Electric of Panasonic Group VBHN240SA11B | Sanyo Electric of Panasonic Group VBMS240AA02 | Sanyo Electric of Panasonic Group VBHN245SA04 | Sanyo Electric of Panasonic Group VBHN245SA04B | Sanyo Electric of Panasonic Group VBHN245SA06 | Sanyo Electric of Panasonic Group VBHN245SA06B | Sanyo Electric of Panasonic Group VBHN245SA11 | Sanyo Electric of Panasonic Group VBHN245SA11B | Sanyo Electric of Panasonic Group VBMS245AA02 | Sanyo Electric of Panasonic Group VBMS250AA02 | Sanyo Electric of Panasonic Group VBMS250AA04 | Sanyo Electric of Panasonic Group VBMS255AA04 | Sanyo Electric of Panasonic Group VBMS260AA04 | Scheuten Solar Logistics P6-60i30-200 | Scheuten Solar Logistics P6-60i30-205 | Scheuten Solar Logistics P6-60i30-210 | Scheuten Solar Logistics P6-60i30-215 | Scheuten Solar Logistics P6-60i30-220 | Scheuten Solar Logistics P6-60i30-225 | Scheuten Solar Logistics P6-60i30-230 | Scheuten Solar Logistics P6-60i30-235 | Scheuten Solar Logistics P6-60i30-240 | Scheuten Solar USA P6-54 185W | Scheuten Solar USA P6-54 190W | Scheuten Solar USA P6-54 195W | Scheuten Solar USA P6-54 200W | Scheuten Solar USA P6-54 205W | Scheuten Solar USA P6-60U-210W | Scheuten Solar USA P6-60U-215W | Scheuten Solar USA P6-60U-220W | Scheuten Solar USA P6-60U-225W | Scheuten Solar USA P6-60U-230W | Scheuten Solar USA P6-60U-235W | Scheuten Solar USA P6-60U-240W | Schuco International MPE 235 PS03 | Schuco International MPE 310 MP 02 | Schuco International MPE 320 MP 02 | Schuco USA MPE 85 AL 01 | Schuco USA MPE 90 AL 01 | Schuco USA S 165-SPU | Schuco USA S 165-SPU-4 | Schuco USA MPE 170 MS 05 | Schuco USA S 170-SPU | Schuco USA S 170-SPU-4 | Schuco USA MPE 175 MS 05 | Schuco USA S 175-SPU-4 | Schuco USA MPE 180 MS 05 | Schuco USA S 180-SPU-4 | Schuco USA MPE 185 MS 05 | Schuco USA MPE 190 MS 05 | Schuco USA MPE 200 PS 04 | Schuco USA SPV 200 SMAU-1 | Schuco USA MPE 205 PS 04 | Schuco USA MPE 210 PS 04 | Schuco USA SPV 210 SMAU-1 | Schuco USA MPE 215 PS 04 | Schuco USA SPV 215 SMAU-1 | Schuco USA MPE 220 PS 04 | Schuco USA MPE 220 PS 09 | Schuco USA SPV 220 SMAU-1 | Schuco USA MPE 225 PS 04 | Schuco USA MPE 225 PS 08 | Schuco USA MPE 225 PS 09 | Schuco USA MPE 225 PS 60 BA | Schuco USA MPE 230 PS 04 | Schuco USA MPE 230 PS 08 | Schuco USA MPE 230 PS 09 | Schuco USA MPE 230 PS 60 BA | Schuco USA MPE 235 PS 08 | Schuco USA MPE 235 PS 09 | Schuco USA MPE 235 PS 60 BA | Schuco USA MPE 240 MS 08 | Schuco USA MPE 240 MS 60 BA | Schuco USA MPE 240 MS 60 BB | Schuco USA MPE 240 PS 08 | Schuco USA MPE 240 PS 09 | Schuco USA MPE 255 PS 60 BA | Schuco USA MPE 245 MS 08 | Schuco USA MPE 245 MS 60 BA | Schuco USA MPE 245 MS 60 BB | Schuco USA MPE 245 PS 08 | Schuco USA MPE 245 PS 60 BA | Schuco USA MPE 250 MS 08 | Schuco USA MPE 250 MS 60 BA | Schuco USA MPE 250 MS 60 BB | Schuco USA MPE 250 PS 60 BA | Schuco USA MPE 240 PS 60 BA | Schuco USA MPE 255 MS 08 | Schuco USA MPE 255 MS 60 BA | Schuco USA MPE 255 MS 60 BB | Schuco USA MPE 260 MS 08 | Schuco USA MPE 260 MS 60 BA | Schuco USA MPE 260 MS 60 BB | Schuco USA MPE 260 PS 60 BA | Schuco USA MPE 265 MS 08 | Schuco USA MPE 265 MS 60 BA | Schuco USA MPE 265 MS 60 BB | Schuco USA MPE 270 MS 08 | Schuco USA MPE 270 MS 60 BA | Schuco USA MPE 270 MS 60 BB | Schuco USA MPE 350 AL 01 | Schuco USA MPE 360 AL 01 | Semyung Electric SM-T-390-Platinum | Semyung Electric SM-T-395-Platinum | Semyung Electric SM-T-400-Platinum | Semyung Electric SM-T-405-Platinum | Semyung Electric SM-T-410-Platinum | S-Energy SM-200MC1 | S-Energy SM-205MC1 | S-Energy SM-210MC1 | S-Energy SM-215MC1 | S-Energy SM-215PC5 | S-Energy SM-220MC1 | S-Energy SM-220PC5 | S-Energy SM-225MC1 | S-Energy SM-225PC5 | S-Energy SM-230MC1 | S-Energy SM-230PC5 | S-Energy SM-230PC8 | S-Energy SM-235MC1 | S-Energy SM-235PC5 | S-Energy SM-235PC8 | S-Energy SM-240PC8 | S-Energy SM-245PC8 | S-Energy SM-250PC8 | S-Energy SM-255PC8 | S-Energy SM-265PC5 | S-Energy SM-270PC5 | S-Energy SM-275PC5 | S-Energy SM-275PC8 | S-Energy SM-280PC5 | S-Energy SM-280PC8 | S-Energy SM-285PC5 | S-Energy SM-285PC8 | S-Energy SM-290PC8 | S-Energy SM-295PC8 | S-Energy SM-300PC8 | S-Energy SM-305PC8 | Seraphim Solar System SRP-180-5MB | Seraphim Solar System SRP-185-5MB | Seraphim Solar System SRP-190-5MB | Seraphim Solar System SRP-195-5MB | Seraphim Solar System SRP-200-5MB | Seraphim Solar System SRP-230-6PB | Seraphim Solar System SRP-235-6PB | Seraphim Solar System SRP-240-6PB | Seraphim Solar System SRP-275-6PA | Seraphim Solar System SRP-280-6PA | Seraphim Solar System SRP-285-6PA | Seraphim Solar System SRP-290-6PA | SET-Solar SETA-125-150W-72M | SET-Solar SETA-125-155W-72M | SET-Solar SETA-125-160W-72M | SET-Solar SDM-170-(165)-72M | SET-Solar SETA-125-165W-72M | SET-Solar SDM-170-(170)-72M | SET-Solar SETA-125-170W-72M | SET-Solar SDM-170-(175)-72M | SET-Solar SETA-125-175W-72M | SET-Solar SETB-125-175W-72M | SET-Solar SDM-170-(180)-72M | SET-Solar SETA-125-180W-72M | SET-Solar SETB-125-180W-72M | SET-Solar SETD-125-180W-72M | SET-Solar SDM-170-(185)-72M | SET-Solar SETA-125-185W-72M | SET-Solar SETB-125-185W-72M | SET-Solar SETD-125-185W-72M | SET-Solar SETB-156-190W-54P | SET-Solar SETB-156-195W-54P | SET-Solar SETB-156-200W-54P | SET-Solar SETB-156-205W-54P | SET-Solar SETB-156-210W-54P | Shandong Linuo Photovoltaic Hi-Tech LN180(36)M-175 | Shandong Linuo Photovoltaic Hi-Tech LN180(36)M-180 | Shandong Linuo Photovoltaic Hi-Tech LN180(36)M-185 | Shandong Linuo Photovoltaic Hi-Tech LN180(36)M-190 | Shandong Linuo Photovoltaic Hi-Tech LN240(30)P-220 | Shandong Linuo Photovoltaic Hi-Tech LN240(30)P-225 | Shandong Linuo Photovoltaic Hi-Tech LN240(30)P-230 | Shandong Linuo Photovoltaic Hi-Tech LN240(30)P-235 | Shandong Linuo Photovoltaic Hi-Tech LN240(30)P-240 | Shanghai Alex Solar Energy Science & Technology ALM-170D-24 | Shanghai Alex Solar Energy Science & Technology ALM-175D-24 | Shanghai Alex Solar Energy Science & Technology ALM-180D-24 | Shanghai Chaori Solar Energy Science & Technology CRM60S125M-24 | Shanghai Chaori Solar Energy Science & Technology CRM60S125S | Shanghai Chaori Solar Energy Science & Technology CRM85S125M-36 | Shanghai Chaori Solar Energy Science & Technology CRM85S125S | Shanghai Chaori Solar Energy Science & Technology CRM115S125M-48 | Shanghai Chaori Solar Energy Science & Technology CRM115S125S | Shanghai Chaori Solar Energy Science & Technology CRM145S125M-60 | Shanghai Chaori Solar Energy Science & Technology CRM145S125S | Shanghai Chaori Solar Energy Science & Technology CRM175S125M-72 | Shanghai Chaori Solar Energy Science & Technology CRM175S125S | Shanghai Chaori Solar Energy Science & Technology CRM180S125M-72 | Shanghai Chaori Solar Energy Science & Technology CRM185S125M-72 | Shanghai Chaori Solar Energy Science & Technology CRM185S156P-54(T) | Shanghai Chaori Solar Energy Science & Technology CRM190S125M-72 | Shanghai Chaori Solar Energy Science & Technology CRM190S156P-54(T) | Shanghai Chaori Solar Energy Science & Technology CRM195S125M-72 | Shanghai Chaori Solar Energy Science & Technology CRM195S125M-80 | Shanghai Chaori Solar Energy Science & Technology CRM195S125S | Shanghai Chaori Solar Energy Science & Technology CRM195S156P-54(T) | Shanghai Chaori Solar Energy Science & Technology CRM200S156P-54(T) | Shanghai Chaori Solar Energy Science & Technology CRM200S156P-60(T) | Shanghai Chaori Solar Energy Science & Technology CRM205S125M-80 | Shanghai Chaori Solar Energy Science & Technology CRM205S156P-54(T) | Shanghai Chaori Solar Energy Science & Technology CRM205S156P-60(T) | Shanghai Chaori Solar Energy Science & Technology CRM210S125M-80 | Shanghai Chaori Solar Energy Science & Technology CRM210S156P-54(T) | Shanghai Chaori Solar Energy Science & Technology CRM210S156P-60(T) | Shanghai Chaori Solar Energy Science & Technology CRM215S125M-80 | Shanghai Chaori Solar Energy Science & Technology CRM215S156P-54(T) | Shanghai Chaori Solar Energy Science & Technology CRM215S156P-60(T) | Shanghai Chaori Solar Energy Science & Technology CRM220S156P-54(T) | Shanghai Chaori Solar Energy Science & Technology CRM220S156P-60(T) | Shanghai Chaori Solar Energy Science & Technology CRM225S156P-54(T) | Shanghai Chaori Solar Energy Science & Technology CRM225S156P-60(T) | Shanghai Chaori Solar Energy Science & Technology CRM230S156P-54(T) | Shanghai Chaori Solar Energy Science & Technology CRM230S156P-60(T) | Shanghai Chaori Solar Energy Science & Technology CRM235S125M-96 | Shanghai Chaori Solar Energy Science & Technology CRM235S125S | Shanghai Chaori Solar Energy Science & Technology CRM235S156P-60(T) | Shanghai Chaori Solar Energy Science & Technology CRM240S125M-96 | Shanghai Chaori Solar Energy Science & Technology CRM240S156P-60(T) | Shanghai Chaori Solar Energy Science & Technology CRM240S156P-72(T) | Shanghai Chaori Solar Energy Science & Technology CRM245S125M-96 | Shanghai Chaori Solar Energy Science & Technology CRM245S156P-60(T) | Shanghai Chaori Solar Energy Science & Technology CRM245S156P-72(T) | Shanghai Chaori Solar Energy Science & Technology CRM250S125M-96 | Shanghai Chaori Solar Energy Science & Technology CRM250S156P-60(T) | Shanghai Chaori Solar Energy Science & Technology CRM250S156P-72(T) | Shanghai Chaori Solar Energy Science & Technology CRM255S125M-96 | Shanghai Chaori Solar Energy Science & Technology CRM255S156P-60(T) | Shanghai Chaori Solar Energy Science & Technology CRM255S156P-72(T) | Shanghai Chaori Solar Energy Science & Technology CRM260S125M-96 | Shanghai Chaori Solar Energy Science & Technology CRM260S156P-60(T) | Shanghai Chaori Solar Energy Science & Technology CRM260S156P-72(T) | Shanghai Chaori Solar Energy Science & Technology CRM265S125M-96 | Shanghai Chaori Solar Energy Science & Technology CRM265S156P-72(T) | Shanghai Chaori Solar Energy Science & Technology CRM270S156P-72(T) | Shanghai Chaori Solar Energy Science & Technology CRM275S156P-72(T) | Shanghai Chaori Solar Energy Science & Technology CRM280S156P-72(T) | Shanghai Chaori Solar Energy Science & Technology CRM285S156P-72(T) | Shanghai Chaori Solar Energy Science & Technology CRM290S156P-72(T) | Shanghai Chaori Solar Energy Science & Technology CRM295S156P-72(T) | Shanghai Chaori Solar Energy Science & Technology CRM300S156P-72(T) | Shanghai JA Solar Technology JAM5-72-165 | Shanghai JA Solar Technology JAM5-72-170 | Shanghai JA Solar Technology JAM5-72-175 | Shanghai JA Solar Technology JAM5(L)(BK)-72-180-SI | Shanghai JA Solar Technology JAM5(L)-72-180-SI | Shanghai JA Solar Technology JAM5-72-180 | Shanghai JA Solar Technology JAM5(L)(BK)-72-185-SI | Shanghai JA Solar Technology JAM5(L)-72-185-SI | Shanghai JA Solar Technology JAM5-72-185 | Shanghai JA Solar Technology JAM5(L)(BK)-72-190-SI | Shanghai JA Solar Technology JAM5(L)-72-190-SI | Shanghai JA Solar Technology JAM5-72-190 | Shanghai JA Solar Technology JAM5(L)(BK)-72-195-SI | Shanghai JA Solar Technology JAM5(L)-72-195-SI | Shanghai JA Solar Technology JAM5-72-195 | Shanghai JA Solar Technology JAM5(L)(BK)-72-200-SI | Shanghai JA Solar Technology JAM5(L)-72-200-SI | Shanghai JA Solar Technology JAM6-60-200 | Shanghai JA Solar Technology JAP6-60-200 | Shanghai JA Solar Technology JAM5(L)(BK)-72-205-SI | Shanghai JA Solar Technology JAM5(L)-72-205-SI | Shanghai JA Solar Technology JAM6-60-205 | Shanghai JA Solar Technology JAP6-60-205 | Shanghai JA Solar Technology JAM5(L)(BK)-72-210-SI | Shanghai JA Solar Technology JAM5(L)-72-210-SI | Shanghai JA Solar Technology JAM6-60-210 | Shanghai JA Solar Technology JAP6-60-210 | Shanghai JA Solar Technology JAM6-60-215 | Shanghai JA Solar Technology JAP6(BK)-60-215 | Shanghai JA Solar Technology JAP6-60-215 | Shanghai JA Solar Technology JAM6-60-220 | Shanghai JA Solar Technology JAP6(BK)-60-220 | Shanghai JA Solar Technology JAP6-60-220 | Shanghai JA Solar Technology JAM6-60-225 | Shanghai JA Solar Technology JAP6(BK)-60-225 | Shanghai JA Solar Technology JAP6-60-225 | Shanghai JA Solar Technology JAP6-60-225-MP | Shanghai JA Solar Technology JAM6-60-230 | Shanghai JA Solar Technology JAP6(BK)-60-230 | Shanghai JA Solar Technology JAP6-60-230 | Shanghai JA Solar Technology JAP6-60-230-MP | Shanghai JA Solar Technology JAM6-60-235 | Shanghai JA Solar Technology JAM6-60-235-SI | Shanghai JA Solar Technology JAP6(BK)-60-235 | Shanghai JA Solar Technology JAP6-60-235 | Shanghai JA Solar Technology JAP6-60-235-MP | Shanghai JA Solar Technology JAM6-60-240 | Shanghai JA Solar Technology JAM6-60-240-SI | Shanghai JA Solar Technology JAP6(BK)-60-240 | Shanghai JA Solar Technology JAP6-60-240 | Shanghai JA Solar Technology JAP6-60-240-MP | Shanghai JA Solar Technology JAM6-60-245-SI | Shanghai JA Solar Technology JAP6(BK)-60-245 | Shanghai JA Solar Technology JAP6-60-245 | Shanghai JA Solar Technology JAP6-60-245-3BB | Shanghai JA Solar Technology JAP6-60-245-MP | Shanghai JA Solar Technology JAM6-60-250-SI | Shanghai JA Solar Technology JAP6(BK)-60-250 | Shanghai JA Solar Technology JAP6-60-250 | Shanghai JA Solar Technology JAP6-60-250-3BB | Shanghai JA Solar Technology JAP6-60-250-MP | Shanghai JA Solar Technology JAP6-72-250 | Shanghai JA Solar Technology JAM6-60-255-SI | Shanghai JA Solar Technology JAM6-72-255 | Shanghai JA Solar Technology JAP6-60-255-3BB | Shanghai JA Solar Technology JAP6-60-255-MP | Shanghai JA Solar Technology JAP6-72-255 | Shanghai JA Solar Technology JAM6-60-260-SI | Shanghai JA Solar Technology JAM6-72-260 | Shanghai JA Solar Technology JAP6-60-260-3BB | Shanghai JA Solar Technology JAP6-60-260-MP | Shanghai JA Solar Technology JAP6-72-260 | Shanghai JA Solar Technology JAM6-72-265 | Shanghai JA Solar Technology JAP6(BK)-72-265 | Shanghai JA Solar Technology JAP6-60-265-3BB | Shanghai JA Solar Technology JAP6-72-265 | Shanghai JA Solar Technology JAM6-72-270 | Shanghai JA Solar Technology JAP6(BK)-72-270 | Shanghai JA Solar Technology JAP6-72-270 | Shanghai JA Solar Technology JAM6-72-275 | Shanghai JA Solar Technology JAP6(BK)-72-275 | Shanghai JA Solar Technology JAP6-72-275 | Shanghai JA Solar Technology JAP6-72-275-3BB | Shanghai JA Solar Technology JAM6-72-280 | Shanghai JA Solar Technology JAP6(BK)-72-280 | Shanghai JA Solar Technology JAP6(BK)-72-280-MP | Shanghai JA Solar Technology JAP6-72-280 | Shanghai JA Solar Technology JAP6-72-280-3BB | Shanghai JA Solar Technology JAP6-72-280-MP | Shanghai JA Solar Technology JAM6(BK)-72-285-SI | Shanghai JA Solar Technology JAM6-72-285 | Shanghai JA Solar Technology JAM6-72-285-SI | Shanghai JA Solar Technology JAP6(BK)-72-285 | Shanghai JA Solar Technology JAP6(BK)-72-285-MP | Shanghai JA Solar Technology JAP6-72-285 | Shanghai JA Solar Technology JAP6-72-285-3BB | Shanghai JA Solar Technology JAP6-72-285-MP | Shanghai JA Solar Technology JAM6(BK)-72-290-SI | Shanghai JA Solar Technology JAM6-72-290 | Shanghai JA Solar Technology JAM6-72-290-SI | Shanghai JA Solar Technology JAP6(BK)-72-290 | Shanghai JA Solar Technology JAP6(BK)-72-290-MP | Shanghai JA Solar Technology JAP6-72-290 | Shanghai JA Solar Technology JAP6-72-290-3BB | Shanghai JA Solar Technology JAP6-72-290-MP | Shanghai JA Solar Technology JAM6(BK)-72-295-SI | Shanghai JA Solar Technology JAM6-72-295 | Shanghai JA Solar Technology JAM6-72-295-SI | Shanghai JA Solar Technology JAP6(BK)-72-295 | Shanghai JA Solar Technology JAP6(BK)-72-295-MP | Shanghai JA Solar Technology JAP6-72-295 | Shanghai JA Solar Technology JAP6-72-295-3BB | Shanghai JA Solar Technology JAP6-72-295-MP | Shanghai JA Solar Technology JAM6(BK)-72-300-SI | Shanghai JA Solar Technology JAM6-72-300 | Shanghai JA Solar Technology JAM6-72-300-SI | Shanghai JA Solar Technology JAP6(BK)-72-300 | Shanghai JA Solar Technology JAP6(BK)-72-300-MP | Shanghai JA Solar Technology JAP6-72-300 | Shanghai JA Solar Technology JAP6-72-300-3BB | Shanghai JA Solar Technology JAP6-72-300-MP | Shanghai JA Solar Technology JAM6(BK)-72-305-SI | Shanghai JA Solar Technology JAM6-72-305-SI | Shanghai JA Solar Technology JAP6(BK)-72-305-MP | Shanghai JA Solar Technology JAP6-72-305 | Shanghai JA Solar Technology JAP6-72-305-3BB | Shanghai JA Solar Technology JAP6-72-305-MP | Shanghai JA Solar Technology JAM6(BK)-72-310-SI | Shanghai JA Solar Technology JAM6-72-310-SI | Shanghai JA Solar Technology JAP6(BK)-72-310-MP | Shanghai JA Solar Technology JAP6-72-310 | Shanghai JA Solar Technology JAP6-72-310-3BB | Shanghai JA Solar Technology JAP6-72-310-MP | Shanghai JA Solar Technology JAM6(BK)-72-315-SI | Shanghai JA Solar Technology JAM6-72-315-SI | Shanghai JA Solar Technology JAP6(BK)-72-315-MP | Shanghai JA Solar Technology JAP6-72-315 | Shanghai JA Solar Technology JAP6-72-315-3BB | Shanghai JA Solar Technology JAP6-72-315-MP | Shanghai Jinglong Solar Energy JLM160S-I | Shanghai Jinglong Solar Energy JLM165S-I | Shanghai Jinglong Solar Energy JLM170S-I | Shanghai Jinglong Solar Energy JLM175S-I | Shanghai Jinglong Solar Energy JLM180S-I | Shanghai Jinglong Solar Energy JLM185S-I | Shanghai Pubsolar GYS-180C | Shanghai Pubsolar GYS-185C | Shanghai Pubsolar GYS-190C | Shanghai Si-Solar Technologies STPV180 | Shanghai Si-Solar Technologies STPV185 | Shanghai Si-Solar Technologies STPV190 | Shanghai Si-Solar Technologies STPV220 | Shanghai Si-Solar Technologies STPV225 | Shanghai Si-Solar Technologies STPV230 | Shanghai Si-Solar Technologies STPV235 | Shanghai Si-Solar Technologies STPV240 | Shanghai Si-Solar Technologies STPV265 | Shanghai Si-Solar Technologies STPV270 | Shanghai Si-Solar Technologies STPV275 | Shanghai Si-Solar Technologies STPV280 | Shanghai Si-Solar Technologies STPV285 | Shanghai Solar Energy S&T S-75D-1 | Shanghai Solar Energy S&T S-90C-1 | Shanghai Solar Energy S&T S-125D-1 | Shanghai Solar Energy S&T S-165D-1 | Shanghai Solar Energy S&T S-165D-A-1 | Shanghai Solar Energy S&T S-175C | Shanghai Solar Energy S&T S-180C | Shanghai Solar Energy S&T S-185C | Shanghai Solar Energy S&T S-205C | Shanghai Solar Energy S&T S-215C | Shanghai Solar Energy S&T S-220D | Shanghai Solar Energy S&T S-225C | Shanghai Solar Energy S&T S-230D | Shanghai Solar Energy S&T S-235C | Shanghai Solar Energy S&T S-245C | Shanghai Solar Energy S&T S-270D | Shanghai ST Solar STM160-72 | Shanghai ST Solar STP160-48 | Shanghai ST Solar STM165-72 | Shanghai ST Solar STP165-48 | Shanghai ST Solar STM170-72 | Shanghai ST Solar STP170-48 | Shanghai ST Solar STM175-72 | Shanghai ST Solar STP175-48 | Shanghai ST Solar STM180-72 | Shanghai ST Solar STP180-48 | Shanghai ST Solar STM185-72 | Shanghai ST Solar STP185-48 | Shanghai ST Solar STP185-54 | Shanghai ST Solar STM190-72 | Shanghai ST Solar STP190-48 | Shanghai ST Solar STP190-54 | Shanghai ST Solar STM195-72 | Shanghai ST Solar STP195-48 | Shanghai ST Solar STP195-54 | Shanghai ST Solar STM200-72 | Shanghai ST Solar STP200-48 | Shanghai ST Solar STP200-54 | Shanghai ST Solar STP205-54 | Shanghai ST Solar STM210-96 | Shanghai ST Solar STP210-54 | Shanghai ST Solar STP210-60 | Shanghai ST Solar STP215-54 | Shanghai ST Solar STP215-60 | Shanghai ST Solar STP220-54 | Shanghai ST Solar STP220-60 | Shanghai ST Solar STM225-96 | Shanghai ST Solar STP225-54 | Shanghai ST Solar STP225-60 | Shanghai ST Solar STP230-60 | Shanghai ST Solar STM235-96 | Shanghai ST Solar STP235-60 | Shanghai ST Solar STM240-96 | Shanghai ST Solar STP240-60 | Shanghai ST Solar STM245-96 | Shanghai ST Solar STP245-60 | Shanghai ST Solar STP245-72 | Shanghai ST Solar STM250-96 | Shanghai ST Solar STP250-60 | Shanghai ST Solar STP250-72 | Shanghai ST Solar STM255-104 | Shanghai ST Solar STM255-96 | Shanghai ST Solar STP255-72 | Shanghai ST Solar STM260-104 | Shanghai ST Solar STM260-96 | Shanghai ST Solar STP260-72 | Shanghai ST Solar STM265-104 | Shanghai ST Solar STP265-72 | Shanghai ST Solar STM270-104 | Shanghai ST Solar STP270-72 | Shanghai ST Solar STM275-104 | Shanghai ST Solar STP275-72 | Shanghai ST Solar STM280-104 | Shanghai ST Solar STP280-72 | Shanghai ST Solar STM285-104 | Shanghai ST Solar STP285-72 | Shanghai ST Solar STP290-72 | Shanghai ST Solar STP295-72 | Shanghai ST Solar STP300-72 | Shanghai ST Solar STM325-130 | Shanghai ST Solar STM330-130 | Shanghai ST Solar STM335-130 | Shanghai ST Solar STM340-130 | Shanghai ST Solar STM345-130 | Shanghai ST Solar STM350-130 | Shanghai Topsolar Green Energy TSM72-125M 160W | Shanghai Topsolar Green Energy TSM72-125M 165W | Shanghai Topsolar Green Energy TSM72-125M 170W | Shanghai Topsolar Green Energy TSM72-125M 175W | Shanghai Topsolar Green Energy TSM72-125M 180W | Shanghai Topsolar Green Energy TSM72-125M 185W | Shanghai Topsolar Green Energy TSM48-156M 190W | Shanghai Topsolar Green Energy TSM72-125M 190W | Shanghai Topsolar Green Energy TSM48-156M 195W | Shanghai Topsolar Green Energy TSM72-125M 195W | Shanghai Topsolar Green Energy TSM48-156M 200W | Shanghai Topsolar Green Energy TSM48-156M 205W | Shanghai Topsolar Green Energy TSM60-156M 210W | Shanghai Topsolar Green Energy TSM60-156M 235W | Shanghai Topsolar Green Energy TSM60-156M 240W | Shanghai Topsolar Green Energy TSM96-125M 240W | Shanghai Topsolar Green Energy TSM60-156M 245W | Shanghai Topsolar Green Energy TSM96-125M 245W | Shanghai Topsolar Green Energy TSM60-156M 250W | Shanghai Topsolar Green Energy TSM96-125M 250W | Shanghai Topsolar Green Energy TSM60-156M 255W | Shanghai Topsolar Green Energy TSM96-125M 255W | Shanghai Topsolar Green Energy TSM96-125M 260W | Shanghai Topsolar Green Energy TSM72-156M 280W | Shanghai Topsolar Green Energy TSM72-156M 285W | Shanghai Topsolar Green Energy TSM72-156M 290W | Shanghai Topsolar Green Energy TSM72-156M 295W | Shanghai Topsolar Green Energy TSM72-156M 300W | Shanghai Topsolar Green Energy TSM72-156M 305W | Shangpin Solar SPSM-175D | Shangpin Solar SPSM-180D | Shangpin Solar SPSM-185D | Shangpin Solar SPSM-215P | Shangpin Solar SPSM-220P | Shangpin Solar SPSM-225D | Shangpin Solar SPSM-225P | Shangpin Solar SPSM-230D | Shangpin Solar SPSM-230P | Shangpin Solar SPSM-235D | Shangpin Solar SPSM-235P | Shangpin Solar SPSM-240D | Shangpin Solar SPSM-245D | Shangpin Solar SPSM-260D | Shangpin Solar SPSM-265D | Shangpin Solar SPSM-270D | Shangpin Solar SPSM-275D | Shangpin Solar SPSM-280D | Shangpin Solar SPSM-285D | Shangpin Solar SPSM-290D | Sharp ND-62RU1 | Sharp ND-62RU1F | Sharp ND-62RU2 | Sharp ND-62RUC1 | Sharp ND-65RU1F | Sharp ND-65RUC1 | Sharp ND-72ELU | Sharp ND-72ELUC | Sharp ND-72ELUF | Sharp ND-72ERU | Sharp ND-72ERUC | Sharp ND-72ERUF | Sharp ND-V075CL | Sharp ND-V075CR | Sharp NA-V115H1 | Sharp NA-V121H1 | Sharp ND-123UJF | Sharp NA-V128H1 | Sharp ND-130UJF | Sharp NA-V135H1 | Sharp ND-N2ECU | Sharp ND-N2ECUC | Sharp ND-N2ECUF | Sharp NE-160U1 | Sharp ND-162U1F | Sharp ND-162U1Y | Sharp ND-162U2 | Sharp NE-165U1 | Sharp NE-165U5 | Sharp NE-165UC1 | Sharp ND-167U1 | Sharp ND-167U1F | Sharp ND-167U1Y | Sharp ND-167U2 | Sharp ND-167U3A | Sharp ND-167UC1 | Sharp NE-170U1 | Sharp NE-170UC1 | Sharp NT-170U1 | Sharp NT-170UC1 | Sharp NT-175U1 | Sharp NT-175UC1 | Sharp ND-176U1Y | Sharp ND-176UC1 | Sharp NT-180U1 | Sharp NU-U180FC | Sharp ND-181U1 | Sharp ND-181U1F | Sharp ND-181U2 | Sharp ND-187U1 | Sharp ND-187U1F | Sharp ND-187U2 | Sharp ND-187UC1 | Sharp ND-198U1F | Sharp ND-198UC1 | Sharp ND-200U1 | Sharp ND-200U1F | Sharp ND-200U2 | Sharp ND-200UC1 | Sharp ND-208U1 | Sharp ND-208U1F | Sharp ND-208U2 | Sharp ND-208UC1 | Sharp ND-208UCJ | Sharp NU-U208FC | Sharp ND-216QCJ | Sharp ND-216U1F | Sharp ND-216U2 | Sharp ND-216UC1 | Sharp ND-216UCJ | Sharp ND-U216C1 | Sharp ND-220U1F | Sharp ND-220UC1 | Sharp ND-220UCJ | Sharp ND-224QCJ | Sharp ND-224U1F | Sharp ND-224UC1 | Sharp ND-224UCJ | Sharp ND-U224C1 | Sharp ND-230QCJ | Sharp ND-230UC1 | Sharp ND-230UCJ | Sharp ND-F2Q230 | Sharp ND-H230Q2 | Sharp ND-L230Q1 | Sharp ND-L230Q2 | Sharp ND-Q230C5 | Sharp ND-Q230F4 | Sharp ND-Q230Q2 | Sharp ND-U230C1 | Sharp ND-U230Q1 | Sharp ND-U230Q2 | Sharp ND-V230A1 | Sharp NU-Q230F4 | Sharp NU-U230F3 | Sharp NU-U230F4 | Sharp ND-235QCJ | Sharp ND-F2Q235 | Sharp ND-H235Q2 | Sharp ND-L235Q1 | Sharp ND-L235Q2 | Sharp ND-Q235C5 | Sharp ND-Q235F4 | Sharp ND-Q235Q2 | Sharp ND-U235Q1 | Sharp ND-U235Q2 | Sharp NU-Q235F2 | Sharp NU-Q235F4 | Sharp NU-U235F1 | Sharp NU-U235F2 | Sharp NU-U235F3 | Sharp NU-U235F4 | Sharp ND-240QCJ | Sharp ND-F5Q240 | Sharp ND-H240Q2 | Sharp ND-L240Q2 | Sharp ND-Q240Q2 | Sharp ND-U240Q2 | Sharp NU-Q240F2 | Sharp NU-Q240W4 | Sharp NU-U240F1 | Sharp NU-U240F2 | Sharp NU-U240P1 | Sharp NU-U240P2 | Sharp ND-245QCJ | Sharp ND-245QCS | Sharp ND-F5Q245 | Sharp ND-H245Q2 | Sharp ND-L245Q2 | Sharp ND-Q245F7 | Sharp ND-Q245Q2 | Sharp ND-U245Q2 | Sharp NU-Q245F2 | Sharp NU-Q245W2 | Sharp NU-Q245W4 | Sharp NU-U245P1 | Sharp NU-U245P2 | Sharp ND-250QCS | Sharp ND-Q250F7 | Sharp NU-Q250W2 | Sharp NU-Q250W4 | Sharp ND-F4Q295 | Sharp ND-F4Q300 | Shenzhen Topray Solar TPS107S-175W(48) | Shenzhen Topray Solar TPS105S-180W(48) | Shenzhen Topray Solar TPS107S-180W(48) | Shenzhen Topray Solar TPS105S-185W(48) | Shenzhen Topray Solar TPS107S-185W(48) | Shenzhen Topray Solar TPS105S-190W(48) | Shenzhen Topray Solar TPS107S-190W(54) | Shenzhen Topray Solar TPS107S-195W(54) | Shenzhen Topray Solar TPS105S-200W(54) | Shenzhen Topray Solar TPS107S-200W(54) | Shenzhen Topray Solar TPS105S-205W(54) | Shenzhen Topray Solar TPS107S-205W(54) | Shenzhen Topray Solar TPS105S-210W(54) | Shenzhen Topray Solar TPS107S-210W(54) | Shenzhen Topray Solar TPS105S-215W(54) | Shenzhen Topray Solar TPS107S-215W(60) | Shenzhen Topray Solar TPS105S-220W(54) | Shenzhen Topray Solar TPS107S-220W(60) | Shenzhen Topray Solar TPS107S-225W(60) | Shenzhen Topray Solar TPS105S-230W(60) | Shenzhen Topray Solar TPS107S-230W(60) | Shenzhen Topray Solar TPS105S-235W(60) | Shenzhen Topray Solar TPS105S-240W(60) | Shenzhen Topray Solar TPS105S-245W(60) | Shenzhen Topray Solar TPS105S-250W(60) | Shenzhen Topray Solar TPS107S-260W(72) | Shenzhen Topray Solar TPS107S-265W(72) | Shenzhen Topray Solar TPS107S-270W(72) | Shenzhen Topray Solar TPS107S-275W(72) | Shenzhen Topray Solar TPS105S-280W(72) | Shenzhen Topray Solar TPS107S-280W(72) | Shenzhen Topray Solar TPS105S-285W(72) | Shenzhen Topray Solar TPS105S-290W(72) | Shenzhen Topray Solar TPS105S-295W(72) | Shenzhen Topray Solar TPS105S-300W(72) | Shenzhen Zhongjing Solar PWM-170W | Shenzhen Zhongjing Solar PWM-175W | Shenzhen Zhongjing Solar PWM-180W | Shenzhen Zhongjing Solar P6Y-230 | Shenzhen Zhongjing Solar P6Y-235 | Shenzhen Zhongjing Solar P6Y-240 | Shenzhen Zhongjing Solar P6Y-245 | Shenzhen Zhongjing Solar M9X-250 | Shenzhen Zhongjing Solar P6Y-250 | Shenzhen Zhongjing Solar M9X-255 | Shenzhen Zhongjing Solar M9X-260 | Shenzhen Zhongjing Solar M9X-265 | Shenzhen Zhongjing Solar P7Y-270 | Shenzhen Zhongjing Solar P7Y-275 | Shenzhen Zhongjing Solar P7Y-280 | Shenzhen Zhongjing Solar P7Y-285 | Shenzhen Zhongjing Solar P7Y-290 | Shinsung Solar Energy SS-BM245B3 | Shinsung Solar Energy SS-BM250B3 | Shinsung Solar Energy SS-BM255B3 | Shinsung Solar Energy SS-BM260B3 | Shinsung Solar Energy SS-BM265B3 | Shinsung Solar Energy SS-DM290B3 | Shinsung Solar Energy SS-DM295B3 | Shinsung Solar Energy SS-DM300B3 | Shinsung Solar Energy SS-DM305B3 | Shinsung Solar Energy SS-DM310B3 | Shinsung Solar Energy SS-DM315B3 | Shinsung Solar Energy SS-DM320B3 | Silevo Triex R215 | Silevo Triex R215 Black | Silevo Triex R220 | Silevo Triex R220 Black | Silevo Triex R225 | Silevo Triex R225 Black | Silevo Triex R230 | Silevo Triex R230 Black | Silevo Triex R235 | Silevo Triex R235 Black | Silevo Triex U290 | Silevo Triex U290 Black | Silevo Triex U295 | Silevo Triex U295 Black | Silevo Triex U300 | Silevo Triex U300 Black | Silevo Triex U305 | Silevo Triex U305 Black | Silevo Triex U310 | Silevo Triex U310 Black | Silfab SLA245M3A | Silfab SLA250M3A | Silfab SLA255M3A | Silfab SLA260M3A | Silfab SLA265M3A | Silicon Energy SiE-165 | Silicon Energy SiE-170 | Silicon Energy SiE-175 | Silicon Energy SiE-180 | Silicon Energy SiE-185 | Silicon Energy SiE-190 | Silicon Energy SiE-195 | Silicon Energy SiE-200 | Silray SRMA-150WP | Silray SRMA-155WP | Silray SRMA-160WP | Silray SRMA-165WP | Silray SRMA-170WP | Silray API-175M | Silray SRAP-175G6M | Silray SRAP-175G6S | Silray SRMA-175WP | Silray API-180M | Silray SR-180 | Silray SRAP-180G6M | Silray SRAP-180G6S | Silray SRMA-180WP | Silray API-185M | Silray API-185M(72)-XH | Silray SRAP-185G6M | Silray SRAP-185G6S | Silray API-190M(72)-XH | Silray SRAP-190G6M | Silray SRAP-190G6S | Silray SRAP-195G6M | Silray SRAP-195G6S | Silray SRAP-200G6M | Silray SRAP-200G6S | Silray SRAP-205G6M | Silray SRAP-205G6S | Silray SRAP-210G6M | Silray SRAP-210G6S | Silray API-215M | Silray API-220P | Silray API-225M | Silray API-230P | Silray API-230P(60)-XH | Silray API-235M | Silray API-235P(60)-XH | Silray API-270P | Silray API-280M(72)-XH | Sintek Photronic STK-S6C2PE-A | Sintek Photronic STK-S6C1ME-A | Sintek Photronic STK-S6B1PE-A | Sintek Photronic STK-S6B1ME-A | SMX Capital SMX185 | SMX Capital SMX230P | Solar Enertech (Shanghai) SE175-72M | Solar Enertech (Shanghai) SE180-72M | Solar Enertech (Shanghai) SE185-72M | Solar Enertech (Shanghai) SE195-54P | Solar Enertech (Shanghai) SE200-54P | Solar Enertech (Shanghai) SE205-54P | Solar Enertech (Shanghai) SE210-54P | Solar Frontier SC70-US-P | Solar Frontier SF70-US-B | Solar Frontier SF70-US-P | Solar Frontier SC75-US-P | Solar Frontier SF75-US-B | Solar Frontier SF75-US-P | Solar Frontier SC80-US-P | Solar Frontier SF80-US-B | Solar Frontier SF80-US-P | Solar Frontier SF85-US-B | Solar Frontier SF85-US-P | Solar Frontier SF90-US-B | Solar Frontier SF130-L | Solar Frontier SF130-M | Solar Frontier SF130-S | Solar Frontier SF130-T | Solar Frontier SF135-L | Solar Frontier SF135-M | Solar Frontier SF135-S | Solar Frontier SF135-T | Solar Frontier SF140-L | Solar Frontier SF140-M | Solar Frontier SF140-S | Solar Frontier SF140-T | Solar Frontier SF145-L | Solar Frontier SF145-M | Solar Frontier SF145-S | Solar Frontier SF145-T | Solar Frontier SF150-L | Solar Frontier SF150-M | Solar Frontier SF150-S | Solar Frontier SF150-T | Solar Frontier SF155-L | Solar Frontier SF155-M | Solar Frontier SF155-S | Solar Frontier SF155-T | Solar Frontier SF160-S | Solar Frontier SF165-S | Solar Frontier SF170-S | Solar Liberty SLX120P6-18 | Solar Liberty SLX125P6-18 | Solar Liberty SLX130P6-18 | Solar Liberty SLX135P6-18 | Solar Liberty SLX140P6-18 | Solar Liberty SLX200P6-30 | Solar Liberty SLX205P6-30 | Solar Liberty SLX210P6-30 | Solar Liberty SLX215P6-30 | Solar Liberty SLX220P6-30 | Solar Liberty SLX225P6-30 | Solar Liberty SLX230P6-30 | Solar Liberty SLX 235 USB | Solar Liberty SLX 235 USC | Solar Liberty SLX 235 USD | Solar Liberty SLX235P6-30 | Solar Liberty SLX 240 USC | Solar Liberty SLX 240 USD | Solar Liberty SLX240P6-36 | Solar Liberty SLX 245 USC | Solar Liberty SLX245P6-36 | Solar Liberty SLX 250 USB | Solar Liberty SLX 250 USC | Solar Liberty SLX 250 USD | Solar Liberty SLX250P6-36 | Solar Liberty SLX 255 USB | Solar Liberty SLX 255 USC | Solar Liberty SLX 255 USD | Solar Liberty SLX255P6-36 | Solar Liberty SLX 260 USB | Solar Liberty SLX 260 USC | Solar Liberty SLX 260 USD | Solar Liberty SLX260P6-36 | Solar Liberty SLX 265 USB | Solar Liberty SLX 265 USC | Solar Liberty SLX 265 USD | Solar Liberty SLX 265 USMB | Solar Liberty SLX 265 USMC | Solar Liberty SLX 265 USMD | Solar Liberty SLX265P6-36 | Solar Liberty SLX 270 USB | Solar Liberty SLX 270 USC | Solar Liberty SLX 270 USD | Solar Liberty SLX 270 USMC | Solar Liberty SLX 270 USMD | Solar Liberty SLX270P6-36 | Solar Liberty SLX275P6-36 | Solar Liberty SLX280P6-36 | Solar Liberty SLX285P6-36 | Solar Liberty SLX 290 USMC | Solar Liberty SLX 290 USMD | Solar Liberty SLX 295 USMC | Solar Liberty SLX 295 USMD | Solar Liberty SLX 300 USMC | Solar Liberty SLX 300 USMD | Solar Liberty SLX 305 USMC | Solar Liberty SLX 305 USMD | Solar Liberty SLX 310 USC | Solar Liberty SLX 310 USMC | Solar Liberty SLX 310 USMD | Solar Liberty SLX 315 USMC | Solar Liberty SLX 315 USMD | Solar Liberty SLX 320 USC | Solar Liberty SLX 320 USMC | Solar Liberty SLX 320 USMD | Solar Liberty SLX 325 USC | Solar Liberty SLX 325 USMC | Solar Liberty SLX 325 USMD | Solar Liberty SLX 330 USC | Solar Liberty SLX 330 USMC | Solar Liberty SLX 330 USMD | Solar Power Industries SPI-M160-60 | Solar Power Industries SPI-M170-60 | Solar Power Industries SPI-M180-60 | Solar Power Industries SPI-M190-60 | Solar Power Industries SPI-156-200W | Solar Power Industries SPI-M200-60 | Solar Power Industries SPI-M210-60 | Solar Power Industries SPI-M215-60 | Solar Power Industries SPI-M220-60 | Solar Power Industries SPI-M220W-60IM | Solar Power Industries SPI-M225-60 | Solar Power Industries SPI-M230-60 | Solar Power Industries SPI-M230W-60IM | Solar Power Industries SPI-M240W-60IM | Solar Semiconductor SSI-S6-125 | Solar Semiconductor SSI-S6-130 | Solar Semiconductor SSI-S6-135 | Solar Semiconductor SSI-S6-140 | Solar Semiconductor SSI-S6-145 | Solar Semiconductor SSI-S6-170 | Solar Semiconductor SSI-S6-175 | Solar Semiconductor SSI-S6-180 | Solar Semiconductor SSI-S6-185 | Solar Semiconductor SSI-S6-190 | Solar Semiconductor SSI-S6-195 | Solar Semiconductor SSI-S6-200 | Solar Semiconductor SSI-S6-205 | Solar Semiconductor SSI-S6-210 | Solar Semiconductor SSI-3M6-215 | Solar Semiconductor SSI-M6-215 | Solar Semiconductor SSI-S6-215 | Solar Semiconductor SSI-3M6-220 | Solar Semiconductor SSI-M6-220 | Solar Semiconductor SSI-S6-220 | Solar Semiconductor SSI-3M6-225 | Solar Semiconductor SSI-M6-225 | Solar Semiconductor SSI-S6-225 | Solar Semiconductor SSI-3M6-230 | Solar Semiconductor SSI-M6-230 | Solar Semiconductor SSI-S6-230 | Solar Semiconductor SSI-3M6-235 | Solar Semiconductor SSI-M6-235 | Solar Semiconductor SSI-S6-235 | Solar Semiconductor SSI-S6-260 | Solar Semiconductor SSI-S6-265 | Solar Semiconductor SSI-S6-270 | Solar Semiconductor SSI-S6-275 | Solar Semiconductor SSI-S6-280 | Solarbest Energy-Tech (Zhejiang) SE-M170(125) | Solarbest Energy-Tech (Zhejiang) ZSB-M170(125) | Solarbest Energy-Tech (Zhejiang) SE-M175(125) | Solarbest Energy-Tech (Zhejiang) ZSB-M175(125) | Solarbest Energy-Tech (Zhejiang) SE-M180(125) | Solarbest Energy-Tech (Zhejiang) ZSB-M180(125) | Solarbest Energy-Tech (Zhejiang) SE-M185(125) | Solarbest Energy-Tech (Zhejiang) ZSB-M185(125) | Solarbest Energy-Tech (Zhejiang) SE-M190(125) | Solarbest Energy-Tech (Zhejiang) ZSB-M190(125) | Solarbest Energy-Tech (Zhejiang) SE-M195(125) | Solarbest Energy-Tech (Zhejiang) ZSB-M195(125) | Solarbest Energy-Tech (Zhejiang) SE-M200(125) | Solarbest Energy-Tech (Zhejiang) ZSB-M200(125) | Solarbest Energy-Tech (Zhejiang) SE-M205(125) | Solarbest Energy-Tech (Zhejiang) ZSB-M205(125) | Solarbest Energy-Tech (Zhejiang) SE-M220(125) | Solarbest Energy-Tech (Zhejiang) SE-M220(156) | Solarbest Energy-Tech (Zhejiang) SE-P220(156) | Solarbest Energy-Tech (Zhejiang) ZSB-M220(125) | Solarbest Energy-Tech (Zhejiang) ZSB-M220(156) | Solarbest Energy-Tech (Zhejiang) ZSB-P220(156) | Solarbest Energy-Tech (Zhejiang) SE-M225(125) | Solarbest Energy-Tech (Zhejiang) SE-M225(156) | Solarbest Energy-Tech (Zhejiang) SE-P225(156) | Solarbest Energy-Tech (Zhejiang) ZSB-M225(125) | Solarbest Energy-Tech (Zhejiang) ZSB-M225(156) | Solarbest Energy-Tech (Zhejiang) ZSB-P225(156) | Solarbest Energy-Tech (Zhejiang) SE-M230(125) | Solarbest Energy-Tech (Zhejiang) SE-M230(156) | Solarbest Energy-Tech (Zhejiang) SE-P230(156) | Solarbest Energy-Tech (Zhejiang) ZSB-M230(125) | Solarbest Energy-Tech (Zhejiang) ZSB-M230(156) | Solarbest Energy-Tech (Zhejiang) ZSB-P230(156) | Solarbest Energy-Tech (Zhejiang) SE-M235(125) | Solarbest Energy-Tech (Zhejiang) SE-M235(156) | Solarbest Energy-Tech (Zhejiang) SE-P235(156) | Solarbest Energy-Tech (Zhejiang) ZSB-M235(125) | Solarbest Energy-Tech (Zhejiang) ZSB-M235(156) | Solarbest Energy-Tech (Zhejiang) ZSB-P235(156) | Solarbest Energy-Tech (Zhejiang) SE-M240(125) | Solarbest Energy-Tech (Zhejiang) SE-M240(156) | Solarbest Energy-Tech (Zhejiang) SE-P240(156) | Solarbest Energy-Tech (Zhejiang) ZSB-M240(125) | Solarbest Energy-Tech (Zhejiang) ZSB-M240(156) | Solarbest Energy-Tech (Zhejiang) ZSB-P240(156) | Solarbest Energy-Tech (Zhejiang) SE-M245(125) | Solarbest Energy-Tech (Zhejiang) SE-M245(156) | Solarbest Energy-Tech (Zhejiang) SE-P245(156) | Solarbest Energy-Tech (Zhejiang) ZSB-M245(125) | Solarbest Energy-Tech (Zhejiang) ZSB-M245(156) | Solarbest Energy-Tech (Zhejiang) ZSB-P245(156) | Solarbest Energy-Tech (Zhejiang) SE-M250(125) | Solarbest Energy-Tech (Zhejiang) SE-M250(156) | Solarbest Energy-Tech (Zhejiang) SE-P250(156) | Solarbest Energy-Tech (Zhejiang) ZSB-M250(125) | Solarbest Energy-Tech (Zhejiang) ZSB-M250(156) | Solarbest Energy-Tech (Zhejiang) ZSB-P250(156) | Solarbest Energy-Tech (Zhejiang) SE-M255(125) | Solarbest Energy-Tech (Zhejiang) SE-M255(156) | Solarbest Energy-Tech (Zhejiang) SE-P255(156) | Solarbest Energy-Tech (Zhejiang) ZSB-M255(125) | Solarbest Energy-Tech (Zhejiang) ZSB-M255(156) | Solarbest Energy-Tech (Zhejiang) ZSB-P255(156) | Solarbest Energy-Tech (Zhejiang) SE-M260(125) | Solarbest Energy-Tech (Zhejiang) SE-M260(156) | Solarbest Energy-Tech (Zhejiang) SE-P260(156) | Solarbest Energy-Tech (Zhejiang) ZSB-M260(125) | Solarbest Energy-Tech (Zhejiang) ZSB-M260(156) | Solarbest Energy-Tech (Zhejiang) ZSB-P260(156) | Solarbest Energy-Tech (Zhejiang) SE-M265(125) | Solarbest Energy-Tech (Zhejiang) SE-M265(156) | Solarbest Energy-Tech (Zhejiang) SE-P265(156) | Solarbest Energy-Tech (Zhejiang) ZSB-M265(125) | Solarbest Energy-Tech (Zhejiang) ZSB-M265(156) | Solarbest Energy-Tech (Zhejiang) ZSB-P265(156) | Solarbest Energy-Tech (Zhejiang) SE-M270(125) | Solarbest Energy-Tech (Zhejiang) SE-M270(156) | Solarbest Energy-Tech (Zhejiang) SE-P270(156) | Solarbest Energy-Tech (Zhejiang) ZSB-M270(125) | Solarbest 